simulink model "acf_force_control_simple"  (R2026b)
settings: Solver=ode4  StopTime=4  FixedStep=1.0000000000000001e-05
InitFcn:
  | acf_select_actuator(bdroot);
model workspace (MAT data in the model file):
  acfControlVersion = 'inertial-delivery-v8'
  acfImplementation = 'simple'
  acfLayoutVersion = 1
  p.actuator.kind = 'voice_coil'
  p.sim.step = 1e-05
  p.sim.stopTime = 4
  p.sim.evaluateFrom = 0
  p.force.reference = 50
  p.force.tolerance = 0.5
  p.force.sampleTime = 0.0001
  p.force.antiWindupRate = 30
  p.force.derivativeFilter = 0.001
  p.force.feedforwardEnabled = 1
  p.mechanics.mA = 0.4
  p.mechanics.mB = 0.6
  p.mechanics.mS = 2
  p.mechanics.k1 = 19746
  p.mechanics.k2 = 19746
  p.mechanics.c1 = 60
  p.mechanics.c2 = 0
  p.mechanics.gravity = 9.81
  p.mechanics.angle = 1.57079632679
  p.mechanics.travelMin = 0
  p.mechanics.travelMax = 0.025
  p.mechanics.midTravel = 0.0125
  p.mechanics.lowerRigid = 0
  p.mechanics.upperRigid = 1
  p.mechanics.externalLowerSpringPair = 1
  p.mechanics.externalUpperSpringPair = 0
  p.robot.initialExcessForce = 10
  p.robot.sampleTime = 0.01
  p.robot.delay = 0.08
  p.robot.recenterGain = 0.8
  p.robot.deadband = 0.0005
  p.robot.responseTime = 0.06
  p.robot.maxSpeed = 0.02
  p.robot.maxAcceleration = 0.5
  p.robot.nominalVelocity = 0.005
  p.robot.errorRiseTime = 0.2
  p.robot.errorForce = 20
  p.robot.forceGate.enabled = 1
  p.robot.forceGate.errorBand_N = 0.2
  p.robot.forceGate.maxRate_N_s = 2
  p.robot.forceGate.dwellTime = 0.1
  p.robot.forceGate.filterTime = 0.1
  p.robot.forceGate.maxDelayGainProduct = 0.25
  p.robot.forceGate.variation.enabled = 1
  p.robot.forceGate.variation.meanTime = 0.1
  p.robot.forceGate.variation.varianceTime = 0.02
  p.robot.forceGate.variation.rmsLimit_N = 0.08
  p.robot.initialPositionOffset_m = 0
  p.sensor.sampleTime = 1e-05
  p.sensor.filterTime = 0.0001
  p.sensor.delay = 2e-05
  p.sensor.bias = 0
  p.sensor.noiseRms = 0.02
  p.sensor.seed = 7
  p.sensor.strokeNoiseRms = 1e-06
  p.sensor.strokeDelay = 2e-05
  p.sensor.distalMass_kg = 2
  p.sensor.distalMass_model_kg = 2
  p.sensor.strokeBias = 0
  p.sensor.positionTarget = 'tool_relative_A'
  p.sensor.positionModel = 1
  p.sensor.distalMassCalibrationScale = 1
  p.sensor.lateralDelayOffsetSamples = 0
  p.sensor.strokeDelayOffset_s = 0
  p.surface.kind = 'sharp_bump'
  p.surface.startTime = 2
  p.surface.height = 0.001
  p.surface.width = 0.01
  p.surface.scanSpeed = 0.1
  p.surface.repeatPeriod = 1.2
  p.screw.lead = 0.01
  p.screw.rotorInertia = 1.58e-06
  p.screw.torqueConstant = 0.0234
  p.screw.backEmfConstant = 0.0234
  p.screw.resistance = 2.32
  p.screw.inductance = 0.000238
  p.screw.peakCurrent = 5
  p.screw.voltage = 24
  p.screw.currentResponse = 0.0001
  p.screw.coulombTorque = 0.001
  p.screw.viscousTorque = 1e-06
  p.screw.frictionSpeed = 1
  p.screw.speedBandwidth = 1000
  p.screw.speedDamping = 0.9
  p.screw.speedAntiWindup = 1000
  p.screw.maxLinearSpeedRequest = 0.1
  p.screw.forceKp = 0.0005
  p.screw.forceKi = 0.005
  p.screw.forceKd = 0
  p.screw.motorReference = 'maxon RE25 302005 (NRND): winding reference only'
  p.screw.motorRotorInertia_kg_m2 = 1.08e-06
  p.screw.screwCouplerInertia_kg_m2 = 5e-07
  p.screw.motorMass_kg = 0.13
  p.screw.continuousCurrent_A = 1.16
  p.screw.continuousTorque_Nm = 0.0263
  p.screw.sizingEfficiency = 0.9
  p.screw.currentDerivativeFilter = 0.0003
  p.screw.currentNotch.enabled = 0
  p.screw.currentNotch.frequency_Hz = 20.2167690051
  p.screw.currentNotch.zeroDamping = 0.01
  p.screw.currentNotch.poleDamping = 0.3
  p.screw.feedbackFilter.kind = 'common'
  p.screw.feedbackFilter.zeroDamping = 0.01
  p.screw.feedbackFilter.poleDamping = 0.3
  p.screw.accelerationPrediction_s = 0
  p.screw.accelerationDerivativeFilter_s = 0.0003
  p.screw.accelerationFeedforwardFilter_s = 0
  p.screw.controlStrategy = 'current'
  p.screw.velocityFeedforwardScale = 0
  p.screw.currentForceKp = 0.408089597672
  p.screw.currentForceKi = 27.2059731781
  p.screw.currentForceKd = 0
  p.coil.forceConstant = 20
  p.coil.resistance = 4
  p.coil.inductance = 0.003
  p.coil.peakCurrent = 3.5
  p.coil.voltage = 24
  p.coil.currentResponse = 0.0001
  p.coil.coulombForce = 0.2
  p.coil.viscousFriction = 2
  p.coil.frictionSpeed = 0.0002
  p.coil.strategy = 'pi'
  p.ideal.positionGain = 100
  p.ideal.velocityTime = 0.005
  p.ideal.maxSpeed = 0.1
  p.ideal.maxAcceleration = 20
  p.ideal.maxAxialForce = Inf
  p.ideal.forceKp = 7.49999999996e-05
  p.ideal.forceKi = 0.0179999999999
  p.ideal.forceKd = 0
  p.d.M = 1
  p.d.alpha = 0.4
  p.d.beta = 0.6
  p.d.mu = 0.24
  p.d.g = 6.00689254982e-16
  p.d.keq = 19746
  p.d.ell = 0.00159154943092
  p.d.q10 = 50
  p.d.q20 = 50
  p.d.holdForce = 50
  p.d.r0 = -0.000506431682366
  p.d.u0 = -0.000506431682366
  p.d.z0 = -0.000202572672946
  p.d.forceTicks = 10
  p.d.sensorTicks = 1
  p.d.robotTicks = 1000
  p.d.sensorDelaySamples = 2
  p.d.robotDelaySamples = 800
  p.d.strokeDelaySamples = 2
  p.d.duration = 0.1
  p.d.screwHoldCurrent = 3.40074664726
  p.d.coilHoldCurrent = 2.5
  p.d.speedKp = 0
  p.d.speedKi = 0
  p.d.forceKp = 0.3
  p.d.forceKi = 20
  p.d.forceFeedforward = 2.5
  p.d.commandMax = 3.5
  p.d.commandMin = -3.5
  p.d.recenterGain = 0.735294117647
  p.d.positionMeasurementBias = -0.0130064316824
  p.d.positionMeasurementInitial = 0.0130064316824
  p.d.forceKd = 0
  p.d.derivativeFilter = 0.001
  p.d.toolMotionObserver.A = [0.950360913569  0.0001; -6.16009725429  1]
  p.d.toolMotionObserver.B = [0.0496390864311  5e-09  -5e-09; 6.16009725429  0.0001  -0.0001]
  p.d.toolMotionObserver.C = [0.950976923294  0; -6.16009725429  1]
  p.d.toolMotionObserver.D = [0.0490230767057  0  0; 6.16009725429  0  0]
  p.d.currentNotch.numerator = [1 0 0]
  p.d.currentNotch.denominator = [1 0 0]
  p.d.currentNotch.initialStates = [2.5; 2.5]
  p.d.feedbackFilter.numerator = [0.0674552738891 0.134910547778 0.0674552738891]
  p.d.feedbackFilter.denominator = [1 -1.14298050254 0.412801598096]
  p.d.feedbackFilter.initialStates = [0; 0]
  p.d.variationGate.meanNumerator = [0.000999500166625 0]
  p.d.variationGate.meanDenominator = [1 -0.999000499833]
  p.d.variationGate.varianceNumerator = [0.00498752080732 0]
  p.d.variationGate.varianceDenominator = [1 -0.995012479193]
  p.d.variationGate.dwellSamples = 1001
  p.d.accelerationPrediction.derivativeNumerator = [2834.68689426 -2834.68689426]
  p.d.accelerationPrediction.derivativeDenominator = [1 -0.716531310574]
  p.d.dragRatio.memoryWeight = 0.980198673307
  p.d.dragRatio.inputWeight = 0.0198013266932
  p.d.positionSampleTime = 1e-05
  p.d.acquisition.numerator = [0.00377324111801 0.00754648223602 0.00377324111801 0]
  p.d.acquisition.denominator = [1 -2.37115334916 1.90670140373 -0.520455090097]
  p.d.acquisition.steadyStatePerUnitInput = [66.2560361718; 66.2560361718; 66.2560361718]
  p.d.acquisition.impulseEnergy = 0.0635425312352
  p.d.acquisition.noiseInputScale = 3.96705064105
  p.d.acquisition.rawSampleTime_s = 1e-05
  p.d.acquisition.nominalLowFrequencyDelay_s = 8.89214154824e-05
  p.d.acquisition.responses.force.numerator = [0.00377324111801 0.00754648223602 0.00377324111801 0]
  p.d.acquisition.responses.force.denominator = [1 -2.37115334916 1.90670140373 -0.520455090097]
  p.d.acquisition.responses.force.steadyStatePerUnitInput = [66.2560361718; 66.2560361718; 66.2560361718]
  p.d.acquisition.responses.force.cutoff_Hz = 5100
  p.d.acquisition.responses.force.emaTime_s = 5e-05
  p.d.acquisition.responses.lateral.numerator = [0.00377324111801 0.00754648223602 0.00377324111801 0]
  p.d.acquisition.responses.lateral.denominator = [1 -2.37115334916 1.90670140373 -0.520455090097]
  p.d.acquisition.responses.lateral.steadyStatePerUnitInput = [66.2560361718; 66.2560361718; 66.2560361718]
  p.d.acquisition.responses.lateral.cutoff_Hz = 5100
  p.d.acquisition.responses.lateral.emaTime_s = 5e-05
  p.d.acquisition.responses.acceleration.numerator = [0.00377324111801 0.00754648223602 0.00377324111801 0]
  p.d.acquisition.responses.acceleration.denominator = [1 -2.37115334916 1.90670140373 -0.520455090097]
  p.d.acquisition.responses.acceleration.steadyStatePerUnitInput = [66.2560361718; 66.2560361718; 66.2560361718]
  p.d.acquisition.responses.acceleration.cutoff_Hz = 5100
  p.d.acquisition.responses.acceleration.emaTime_s = 5e-05
  p.d.acquisition.responses.position.numerator = [0.00377324111801 0.00754648223602 0.00377324111801 0]
  p.d.acquisition.responses.position.denominator = [1 -2.37115334916 1.90670140373 -0.520455090097]
  p.d.acquisition.responses.position.steadyStatePerUnitInput = [66.2560361718; 66.2560361718; 66.2560361718]
  p.d.acquisition.responses.position.cutoff_Hz = 5100
  p.d.acquisition.responses.position.emaTime_s = 5e-05
  p.d.acquisition.responses.frame.numerator = [0.00377324111801 0.00754648223602 0.00377324111801 0]
  p.d.acquisition.responses.frame.denominator = [1 -2.37115334916 1.90670140373 -0.520455090097]
  p.d.acquisition.responses.frame.steadyStatePerUnitInput = [66.2560361718; 66.2560361718; 66.2560361718]
  p.d.acquisition.responses.frame.cutoff_Hz = 5100
  p.d.acquisition.responses.frame.emaTime_s = 5e-05
  p.d.acquisition.noiseReferenceImpulseEnergy = 0.0635425312352
  p.d.acquisition.frameDelaySamples = 2
  p.d.acquisition.accelerationNoiseInputScale = 3.96705064105
  p.d.acquisition.positionNoiseInputScale = 3.96705064105
  p.d.actualRobotTransportSampleTime_s = 0.0001
  p.d.preparedScanSpeed_m_s = 0.1
  p.d.preparedSensorDelay_s = 2e-05
  p.d.identifiedHolderMass_kg = 0.6
  p.d.identifiedMovingMass_kg = 2.6
  p.d.coilForceConstant_model_N_A = 20
  p.d.screwTorqueConstant_model_Nm_A = 0.0234
  p.d.coilHoldingCurrentCommand_A = 2.5
  p.d.screwHoldingCurrentCommand_A = 3.40074664726
  p.d.screwMovingMass = 0.6
  p.d.screwAccelerationPrediction.derivativeNumerator = [2834.68689426 -2834.68689426]
  p.d.screwAccelerationPrediction.derivativeDenominator = [1 -0.716531310574]
  p.d.screwAccelerationFeedforwardFilter.numerator = [1 0]
  p.d.screwAccelerationFeedforwardFilter.denominator = [1 0]
  p.d.screwCurrentNotch.numerator = [1 0 0]
  p.d.screwCurrentNotch.denominator = [1 0 0]
  p.d.screwCurrentNotch.initialStates = [3.40074664726; 3.40074664726]
  p.d.screwFeedbackFilter.numerator = [0.0674552738891 0.134910547778 0.0674552738891]
  p.d.screwFeedbackFilter.denominator = [1 -1.14298050254 0.412801598096]
  p.d.screwFeedbackFilter.initialStates = [0; 0]
  p.d.screwLowerLoadInverse.enabled = 1
  p.d.screwLowerLoadInverse.scale = 1
  p.d.screwLowerLoadInverse.cutoff_Hz = 1500
  p.d.screwLowerLoadInverse.filterDamping = 0.707106781187
  p.d.screwLowerLoadInverse.identifiedStiffness_N_m = 19746
  p.d.screwLowerLoadInverse.identifiedDamping_Ns_m = 60
  p.d.screwLowerLoadInverse.identifiedMassB_kg = 1.22375899815
  p.d.screwLowerLoadInverse.numerator = [3.57861341628 -3.57861341628 -3.57861341628 3.57861341628]
  p.d.screwLowerLoadInverse.denominator = [1 -1.71541194562 0.995792771996 -0.263401371553]
  p.d.screwLowerLoadInverse.identifiedForceConstant_N_A = 14.7026536188
  p.d.screwLowerLoadInverse.stiffnessCalibrationScale = 1
  p.d.screwLowerLoadInverse.dampingCalibrationScale = 1
  p.d.screwLowerLoadInverse.dampingCalibrationOffset_Ns_m = 0
  p.robotPrediction.enabled = 1
  p.robotPrediction.delay = 0.08
  p.robotPrediction.responseTime = 0.06
  p.robotPrediction.maxSpeed = 0.02
  p.robotPrediction.maxAcceleration = 0.5
  p.robotPrediction.boundedNominalPath = 1
  p.robotPrediction.delaySamples = 8
  p.robotPrediction.surfaceJerkEnabled = 0
  p.robotPrediction.surfaceSnapPower = 1000000
  p.robotPrediction.surfaceJerkDecayTime = Inf
  p.robotPrediction.surfaceJerkFeedforwardGain = 0
  p.contact.mu = 0.3
  p.contact.lateralNoiseRms_N = 0.02
  p.contact.lateralBias_N = 0
  p.contact.slopeFilterTime_s = 0
  p.contact.normalIntegralScale = 1
  p.contact.geometryFeedforwardScale = 1
  p.contact.lateralPredictionTime_s = 0
  p.contact.lateralDerivativeFilterTime_s = 0.0003
  p.contact.commandedScanSpeed_m_s = 0.1
  p.contact.lateralDelaySamples = 2
  p.contact.geometryMode = 'measured_drag_ratio'
  p.contact.dragRatioFilter_s = 0.005
  p.contact.dragRatioMinForce_N = 1
  p.contact.commandedScanSpeedScale = 1
  p.accel.enabled = 1
  p.accel.filterTime = 0.0001
  p.accel.delay = 2e-05
  p.accel.noiseRms = 0.014
  p.accel.bias = 0
  p.accel.scaleError = 0
  p.accel.range_g = 50
  p.accel.quantum = 0.00468
  p.accel.delaySamples = 2
  p.accel.nominalNoiseRms = 0.014
  p.accel.delayOffset_s = 0
  p.inertial.forceKp = 0.3
  p.inertial.forceKi = 20
  p.inertial.forceKd = 0
  p.inertial.derivativeFilter = 0.001
  p.inertial.positionBandwidth_Hz = 40
  p.inertial.accelerationFeedforwardScale = 1
  p.inertial.guideFrictionFeedforwardScale = 1
  p.inertial.guideVelocityPrediction_s = 0.0004
  p.inertial.currentNotch.enabled = 0
  p.inertial.currentNotch.frequency_Hz = 1643.74518416
  p.inertial.currentNotch.zeroDamping = 0.001
  p.inertial.currentNotch.poleDamping = 1
  p.inertial.feedbackFilter.enabled = 1
  p.inertial.feedbackFilter.cutoff_Hz = 1000
  p.inertial.feedbackFilter.damping = 0.707106781187
  p.inertial.accelerationPrediction_s = 0
  p.inertial.accelerationDerivativeFilter_s = 0.0003
  p.inertial.lowerLoadInverse.enabled = 1
  p.inertial.lowerLoadInverse.scale = 1
  p.inertial.lowerLoadInverse.cutoff_Hz = 1500
  p.inertial.lowerLoadInverse.filterDamping = 0.707106781187
  p.inertial.lowerLoadInverse.identifiedStiffness_N_m = 19746
  p.inertial.lowerLoadInverse.identifiedDamping_Ns_m = 60
  p.inertial.lowerLoadInverse.identifiedMassB_kg = 0.6
  p.inertial.lowerLoadInverse.numerator = [1.28984008064 -1.28984008064 -1.28984008064 1.28984008064]
  p.inertial.lowerLoadInverse.denominator = [1 -1.71541194562 0.995792771996 -0.263401371553]
  p.inertial.lowerLoadInverse.identifiedForceConstant_N_A = 20
  p.inertial.lowerLoadInverse.stiffnessCalibrationScale = 1
  p.inertial.lowerLoadInverse.dampingCalibrationScale = 1
  p.inertial.lowerLoadInverse.dampingCalibrationOffset_Ns_m = 0
  p.inertial.holderMassCalibrationScale = 1
  p.inertial.forceConstantCalibrationScale = 1
  p.sensorDesign.accelerometer = 'Two orthogonal ADXL1002 analog axes'
  p.sensorDesign.noiseDensity_ug_sqrtHz = 25
  p.sensorDesign.assumedENBW_Hz = 3177.12656176
  p.sensorDesign.derivedRMS_m_s2 = 0.0138190421649
  p.sensorDesign.modeledRMS_m_s2 = 0.014
  p.sensorDesign.nominalModeledRMS_m_s2 = 0.014
  p.sensorDesign.ADCbits = 18
  p.sensorDesign.ADCvoltageRange_V = [0 5]
  p.sensorDesign.sensitivity_V_g = 0.04
  p.sensorDesign.derivedQuantum_m_s2 = 0.00467617511749
  p.sensorDesign.modeledQuantum_m_s2 = 0.00468
  p.sensorDesign.modeledRange_g = 50
  p.sensorDesign.rawSampleTime_s = 1e-05
  p.sensorDesign.antiAliasCutoff_Hz = 5100
  p.sensorDesign.antiAliasDamping = 0.707106781187
  p.sensorDesign.conditioningEMA_s = 5e-05
  p.sensorDesign.responseGroupDelay_s = 8.89214154824e-05
  p.sensorDesign.commonAcquisitionDelay_s = 2e-05
  p.sensorDesign.identifiedMotionFrameDelay_s = 2e-05
  p.sensorDesign.forceConditioning = 'Designed common two-pole AA and fresh EMA; actual and identified response/phase are explicit.'
  p.sensorDesign.interpretation = 'Engineered and identified acquisition target, not a guaranteed manufacturer transfer. Noise is conditioned RMS before conservative post-response ADC quantization.'
  p.springs.lower.part = 'Approximate guided spring target; confirm working envelope'
  p.springs.lower.rate_N_m = 9873
  p.springs.lower.freeLength_m = 0.02
  p.springs.lower.freeLengthTolerance_m = 0.00049
  p.springs.lower.minWorkingLength_m = 0.01055
  p.springs.lower.maxCyclicStroke_m = 0.00318
  p.springs.lower.forceEnvelope_N = 68.543
  p.springs.upper.part = 'Approximate guided spring target; confirm working envelope'
  p.springs.upper.rate_N_m = 9873
  p.springs.upper.freeLength_m = 0.02
  p.springs.upper.freeLengthTolerance_m = 0.00049
  p.springs.upper.minWorkingLength_m = 0.01055
  p.springs.upper.maxCyclicStroke_m = 0.00318
  p.springs.upper.forceEnvelope_N = 68.543
  p.springs.commonPreload_N = 33.6
  p.springs.maxCombinedLength_m = 0.1
  p.springs.workingClearance_m = 0.0005
  p.springs.unseatingClearance_m = 0.00025
  p.springs.sensingCell.stiffness_N_m = 64000000
  p.springs.sensingCell.separateNativeState = 0
  p.springs.sensingCell.masslessSeriesApproximation = 1
  p.springs.sensingCell.structuralDampingQualified = 0
  p.springs.sensingCell.loadPath = 'B -> opposed guided spring pair parallel with damper -> joining frame -> multi-axis B-S load cell -> S'
  p.springs.sensingCell.loadCellBypass = 0
  p.springs.sensingCell.prototypeMountModeQualificationRequired = 1
  p.acquisition.enabled = 1
  p.acquisition.rawSampleTime_s = 1e-05
  p.acquisition.antiAliasCutoff_Hz = 5100
  p.acquisition.antiAliasDamping = 0.707106781187
  p.acquisition.emaTime_s = 5e-05
  p.acquisition.pipelineDelay_s = 2e-05
  p.acquisition.forceDelayOffset_s = 0
  p.acquisition.lateralDelayOffset_s = 0
  p.acquisition.accelerationDelayOffset_s = 0
  p.acquisition.positionDelayOffset_s = 0
  p.acquisition.requireFastVariationGate = 1
  p.acquisition.identifiedAntiAliasCutoff_Hz = 5100
  p.acquisition.identifiedEmaTime_s = 5e-05
  p.acquisition.identifiedPipelineDelay_s = 2e-05
  p.acquisition.forceAntiAliasScale = 1
  p.acquisition.lateralAntiAliasScale = 1
  p.acquisition.accelerationAntiAliasScale = 1
  p.acquisition.positionAntiAliasScale = 1
  p.acquisition.motionFrameDelayOffset_s = 0
  pCompliant.actuator.kind = 'voice_coil'
  pCompliant.sim.step = 1e-05
  pCompliant.sim.stopTime = 4
  pCompliant.sim.evaluateFrom = 0
  pCompliant.force.reference = 50
  pCompliant.force.tolerance = 0.5
  pCompliant.force.sampleTime = 0.0001
  pCompliant.force.antiWindupRate = 30
  pCompliant.force.derivativeFilter = 0.001
  pCompliant.force.feedforwardEnabled = 1
  pCompliant.mechanics.mA = 0.4
  pCompliant.mechanics.mB = 0.6
  pCompliant.mechanics.mS = 1.4
  pCompliant.mechanics.k1 = 19746
  pCompliant.mechanics.k2 = 19746
  pCompliant.mechanics.c1 = 30
  pCompliant.mechanics.c2 = 5
  pCompliant.mechanics.gravity = 9.81
  pCompliant.mechanics.angle = 0
  pCompliant.mechanics.travelMin = 0
  pCompliant.mechanics.travelMax = 0.025
  pCompliant.mechanics.midTravel = 0.0125
  pCompliant.mechanics.lowerRigid = 0
  pCompliant.mechanics.upperRigid = 0
  pCompliant.mechanics.externalLowerSpringPair = 1
  pCompliant.mechanics.externalUpperSpringPair = 1
  pCompliant.robot.initialExcessForce = 10
  pCompliant.robot.sampleTime = 0.01
  pCompliant.robot.delay = 0.08
  pCompliant.robot.recenterGain = 0.8
  pCompliant.robot.deadband = 0.0005
  pCompliant.robot.responseTime = 0.06
  pCompliant.robot.maxSpeed = 0.02
  pCompliant.robot.maxAcceleration = 0.5
  pCompliant.robot.nominalVelocity = 0.005
  pCompliant.robot.errorRiseTime = 0.2
  pCompliant.robot.errorForce = 20
  pCompliant.robot.forceGate.enabled = 1
  pCompliant.robot.forceGate.errorBand_N = 0.2
  pCompliant.robot.forceGate.maxRate_N_s = 2
  pCompliant.robot.forceGate.dwellTime = 0.1
  pCompliant.robot.forceGate.filterTime = 0.1
  pCompliant.robot.forceGate.maxDelayGainProduct = 0.25
  pCompliant.robot.forceGate.variation.enabled = 1
  pCompliant.robot.forceGate.variation.meanTime = 0.1
  pCompliant.robot.forceGate.variation.varianceTime = 0.02
  pCompliant.robot.forceGate.variation.rmsLimit_N = 0.08
  pCompliant.robot.initialPositionOffset_m = 0
  pCompliant.sensor.sampleTime = 1e-05
  pCompliant.sensor.filterTime = 0.0001
  pCompliant.sensor.delay = 2e-05
  pCompliant.sensor.bias = 0
  pCompliant.sensor.noiseRms = 0.02
  pCompliant.sensor.seed = 7
  pCompliant.sensor.strokeNoiseRms = 1e-06
  pCompliant.sensor.strokeDelay = 2e-05
  pCompliant.sensor.distalMass_kg = 1.4
  pCompliant.sensor.distalMass_model_kg = 1.4
  pCompliant.sensor.strokeBias = 0
  pCompliant.sensor.positionTarget = 'tool_relative_A'
  pCompliant.sensor.positionModel = 1
  pCompliant.sensor.distalMassCalibrationScale = 1
  pCompliant.sensor.lateralDelayOffsetSamples = 0
  pCompliant.sensor.strokeDelayOffset_s = 0
  pCompliant.surface.kind = 'sharp_bump'
  pCompliant.surface.startTime = 2
  pCompliant.surface.height = 0.001
  pCompliant.surface.width = 0.01
  pCompliant.surface.scanSpeed = 0.1
  pCompliant.surface.repeatPeriod = 1.2
  pCompliant.screw.lead = 0.01
  pCompliant.screw.rotorInertia = 1.58e-06
  pCompliant.screw.torqueConstant = 0.0234
  pCompliant.screw.backEmfConstant = 0.0234
  pCompliant.screw.resistance = 2.32
  pCompliant.screw.inductance = 0.000238
  pCompliant.screw.peakCurrent = 5
  pCompliant.screw.voltage = 24
  pCompliant.screw.currentResponse = 0.0001
  pCompliant.screw.coulombTorque = 0.001
  pCompliant.screw.viscousTorque = 1e-06
  pCompliant.screw.frictionSpeed = 1
  pCompliant.screw.speedBandwidth = 1000
  pCompliant.screw.speedDamping = 0.9
  pCompliant.screw.speedAntiWindup = 1000
  pCompliant.screw.maxLinearSpeedRequest = 0.1
  pCompliant.screw.forceKp = 0.0005
  pCompliant.screw.forceKi = 0.005
  pCompliant.screw.forceKd = 0
  pCompliant.screw.motorReference = 'maxon RE25 302005 (NRND): winding reference only'
  pCompliant.screw.motorRotorInertia_kg_m2 = 1.08e-06
  pCompliant.screw.screwCouplerInertia_kg_m2 = 5e-07
  pCompliant.screw.motorMass_kg = 0.13
  pCompliant.screw.continuousCurrent_A = 1.16
  pCompliant.screw.continuousTorque_Nm = 0.0263
  pCompliant.screw.sizingEfficiency = 0.9
  pCompliant.screw.currentDerivativeFilter = 0.0003
  pCompliant.screw.currentNotch.enabled = 0
  pCompliant.screw.currentNotch.frequency_Hz = 20.2167690051
  pCompliant.screw.currentNotch.zeroDamping = 0.01
  pCompliant.screw.currentNotch.poleDamping = 0.3
  pCompliant.screw.feedbackFilter.kind = 'common'
  pCompliant.screw.feedbackFilter.zeroDamping = 0.01
  pCompliant.screw.feedbackFilter.poleDamping = 0.3
  pCompliant.screw.accelerationPrediction_s = 0
  pCompliant.screw.accelerationDerivativeFilter_s = 0.0003
  pCompliant.screw.accelerationFeedforwardFilter_s = 0
  pCompliant.screw.controlStrategy = 'current'
  pCompliant.screw.velocityFeedforwardScale = 0
  pCompliant.screw.currentForceKp = 0.408089597672
  pCompliant.screw.currentForceKi = 27.2059731781
  pCompliant.screw.currentForceKd = 0
  pCompliant.coil.forceConstant = 20
  pCompliant.coil.resistance = 4
  pCompliant.coil.inductance = 0.003
  pCompliant.coil.peakCurrent = 3.5
  pCompliant.coil.voltage = 24
  pCompliant.coil.currentResponse = 0.0001
  pCompliant.coil.coulombForce = 0.2
  pCompliant.coil.viscousFriction = 2
  pCompliant.coil.frictionSpeed = 0.0002
  pCompliant.coil.strategy = 'pi'
  pCompliant.ideal.positionGain = 100
  pCompliant.ideal.velocityTime = 0.005
  pCompliant.ideal.maxSpeed = 0.1
  pCompliant.ideal.maxAcceleration = 20
  pCompliant.ideal.maxAxialForce = Inf
  pCompliant.ideal.forceKp = 7.49999999996e-05
  pCompliant.ideal.forceKi = 0.0179999999999
  pCompliant.ideal.forceKd = 0
  pCompliant.d.M = 1
  pCompliant.d.alpha = 0.4
  pCompliant.d.beta = 0.6
  pCompliant.d.mu = 0.24
  pCompliant.d.g = 9.81
  pCompliant.d.keq = 9873
  pCompliant.d.ell = 0.00159154943092
  pCompliant.d.q10 = 36.266
  pCompliant.d.q20 = 26.456
  pCompliant.d.holdForce = 30.38
  pCompliant.d.r0 = -0.00101286336473
  pCompliant.d.u0 = -0.00101286336473
  pCompliant.d.z0 = -0.000405145345893
  pCompliant.d.forceTicks = 10
  pCompliant.d.sensorTicks = 1
  pCompliant.d.robotTicks = 1000
  pCompliant.d.sensorDelaySamples = 2
  pCompliant.d.robotDelaySamples = 800
  pCompliant.d.strokeDelaySamples = 2
  pCompliant.d.duration = 0.1
  pCompliant.d.screwHoldCurrent = 2.06629366288
  pCompliant.d.coilHoldCurrent = 1.519
  pCompliant.d.speedKp = 0
  pCompliant.d.speedKi = 0
  pCompliant.d.forceKp = 0.3
  pCompliant.d.forceKi = 20
  pCompliant.d.forceFeedforward = 1.519
  pCompliant.d.commandMax = 3.5
  pCompliant.d.commandMin = -3.5
  pCompliant.d.recenterGain = 0.735294117647
  pCompliant.d.positionMeasurementBias = -0.0135128633647
  pCompliant.d.positionMeasurementInitial = 0.0135128633647
  pCompliant.d.forceKd = 0
  pCompliant.d.derivativeFilter = 0.001
  pCompliant.d.positionSampleTime = 1e-05
  pCompliant.d.actualRobotTransportSampleTime_s = 0.0001
  pCompliant.d.preparedScanSpeed_m_s = 0.1
  pCompliant.d.preparedSensorDelay_s = 2e-05
  pCompliant.d.identifiedHolderMass_kg = 0.6
  pCompliant.d.identifiedMovingMass_kg = 2
  pCompliant.d.coilForceConstant_model_N_A = 20
  pCompliant.d.screwTorqueConstant_model_Nm_A = 0.0234
  pCompliant.d.coilHoldingCurrentCommand_A = 1.519
  pCompliant.d.screwHoldingCurrentCommand_A = 2.06629366288
  pCompliant.d.screwMovingMass = 0.24
  pCompliant.d.screwAccelerationPrediction.derivativeNumerator = [2834.68689426 -2834.68689426]
  pCompliant.d.screwAccelerationPrediction.derivativeDenominator = [1 -0.716531310574]
  pCompliant.d.screwAccelerationFeedforwardFilter.numerator = [1 0]
  pCompliant.d.screwAccelerationFeedforwardFilter.denominator = [1 0]
  pCompliant.d.screwCurrentNotch.numerator = [1 0 0]
  pCompliant.d.screwCurrentNotch.denominator = [1 0 0]
  pCompliant.d.screwCurrentNotch.initialStates = [2.06629366288; 2.06629366288]
  pCompliant.d.screwFeedbackFilter.numerator = [0.0674552738891 0.134910547778 0.0674552738891]
  pCompliant.d.screwFeedbackFilter.denominator = [1 -1.14298050254 0.412801598096]
  pCompliant.d.screwFeedbackFilter.initialStates = [0; 0]
  pCompliant.d.screwLowerLoadInverse.enabled = 1
  pCompliant.d.screwLowerLoadInverse.scale = 1
  pCompliant.d.screwLowerLoadInverse.cutoff_Hz = 1500
  pCompliant.d.screwLowerLoadInverse.filterDamping = 0.707106781187
  pCompliant.d.screwLowerLoadInverse.identifiedStiffness_N_m = 19746
  pCompliant.d.screwLowerLoadInverse.identifiedDamping_Ns_m = 30
  pCompliant.d.screwLowerLoadInverse.identifiedMassB_kg = 1.22375899815
  pCompliant.d.screwLowerLoadInverse.numerator = [7.04320705588 -7.04320705588 -7.04320705588 7.04320705588]
  pCompliant.d.screwLowerLoadInverse.denominator = [1 -1.68406629824 0.972352836098 -0.254868618096]
  pCompliant.d.screwLowerLoadInverse.identifiedForceConstant_N_A = 14.7026536188
  pCompliant.d.screwLowerLoadInverse.stiffnessCalibrationScale = 1
  pCompliant.d.screwLowerLoadInverse.dampingCalibrationScale = 1
  pCompliant.d.screwLowerLoadInverse.dampingCalibrationOffset_Ns_m = 0
  pCompliant.d.currentNotch.numerator = [1 0 0]
  pCompliant.d.currentNotch.denominator = [1 0 0]
  pCompliant.d.currentNotch.initialStates = [1.519; 1.519]
  pCompliant.d.feedbackFilter.numerator = [0.0674552738891 0.134910547778 0.0674552738891]
  pCompliant.d.feedbackFilter.denominator = [1 -1.14298050254 0.412801598096]
  pCompliant.d.feedbackFilter.initialStates = [0; 0]
  pCompliant.d.variationGate.meanNumerator = [0.000999500166625 0]
  pCompliant.d.variationGate.meanDenominator = [1 -0.999000499833]
  pCompliant.d.variationGate.varianceNumerator = [0.00498752080732 0]
  pCompliant.d.variationGate.varianceDenominator = [1 -0.995012479193]
  pCompliant.d.variationGate.dwellSamples = 1001
  pCompliant.d.accelerationPrediction.derivativeNumerator = [2834.68689426 -2834.68689426]
  pCompliant.d.accelerationPrediction.derivativeDenominator = [1 -0.716531310574]
  pCompliant.d.dragRatio.memoryWeight = 0.980198673307
  pCompliant.d.dragRatio.inputWeight = 0.0198013266932
  pCompliant.d.toolMotionObserver.A = [0.950360913569  0.0001; -6.16009725429  1]
  pCompliant.d.toolMotionObserver.B = [0.0496390864311  5e-09  -5e-09; 6.16009725429  0.0001  -0.0001]
  pCompliant.d.toolMotionObserver.C = [0.950976923294  0; -6.16009725429  1]
  pCompliant.d.toolMotionObserver.D = [0.0490230767057  0  0; 6.16009725429  0  0]
  pCompliant.d.acquisition.numerator = [0.00377324111801 0.00754648223602 0.00377324111801 0]
  pCompliant.d.acquisition.denominator = [1 -2.37115334916 1.90670140373 -0.520455090097]
  pCompliant.d.acquisition.steadyStatePerUnitInput = [66.2560361718; 66.2560361718; 66.2560361718]
  pCompliant.d.acquisition.impulseEnergy = 0.0635425312352
  pCompliant.d.acquisition.noiseInputScale = 3.96705064105
  pCompliant.d.acquisition.rawSampleTime_s = 1e-05
  pCompliant.d.acquisition.nominalLowFrequencyDelay_s = 8.89214154824e-05
  pCompliant.d.acquisition.responses.force.numerator = [0.00377324111801 0.00754648223602 0.00377324111801 0]
  pCompliant.d.acquisition.responses.force.denominator = [1 -2.37115334916 1.90670140373 -0.520455090097]
  pCompliant.d.acquisition.responses.force.steadyStatePerUnitInput = [66.2560361718; 66.2560361718; 66.2560361718]
  pCompliant.d.acquisition.responses.force.cutoff_Hz = 5100
  pCompliant.d.acquisition.responses.force.emaTime_s = 5e-05
  pCompliant.d.acquisition.responses.lateral.numerator = [0.00377324111801 0.00754648223602 0.00377324111801 0]
  pCompliant.d.acquisition.responses.lateral.denominator = [1 -2.37115334916 1.90670140373 -0.520455090097]
  pCompliant.d.acquisition.responses.lateral.steadyStatePerUnitInput = [66.2560361718; 66.2560361718; 66.2560361718]
  pCompliant.d.acquisition.responses.lateral.cutoff_Hz = 5100
  pCompliant.d.acquisition.responses.lateral.emaTime_s = 5e-05
  pCompliant.d.acquisition.responses.acceleration.numerator = [0.00377324111801 0.00754648223602 0.00377324111801 0]
  pCompliant.d.acquisition.responses.acceleration.denominator = [1 -2.37115334916 1.90670140373 -0.520455090097]
  pCompliant.d.acquisition.responses.acceleration.steadyStatePerUnitInput = [66.2560361718; 66.2560361718; 66.2560361718]
  pCompliant.d.acquisition.responses.acceleration.cutoff_Hz = 5100
  pCompliant.d.acquisition.responses.acceleration.emaTime_s = 5e-05
  pCompliant.d.acquisition.responses.position.numerator = [0.00377324111801 0.00754648223602 0.00377324111801 0]
  pCompliant.d.acquisition.responses.position.denominator = [1 -2.37115334916 1.90670140373 -0.520455090097]
  pCompliant.d.acquisition.responses.position.steadyStatePerUnitInput = [66.2560361718; 66.2560361718; 66.2560361718]
  pCompliant.d.acquisition.responses.position.cutoff_Hz = 5100
  pCompliant.d.acquisition.responses.position.emaTime_s = 5e-05
  pCompliant.d.acquisition.responses.frame.numerator = [0.00377324111801 0.00754648223602 0.00377324111801 0]
  pCompliant.d.acquisition.responses.frame.denominator = [1 -2.37115334916 1.90670140373 -0.520455090097]
  pCompliant.d.acquisition.responses.frame.steadyStatePerUnitInput = [66.2560361718; 66.2560361718; 66.2560361718]
  pCompliant.d.acquisition.responses.frame.cutoff_Hz = 5100
  pCompliant.d.acquisition.responses.frame.emaTime_s = 5e-05
  pCompliant.d.acquisition.noiseReferenceImpulseEnergy = 0.0635425312352
  pCompliant.d.acquisition.frameDelaySamples = 2
  pCompliant.d.acquisition.accelerationNoiseInputScale = 3.96705064105
  pCompliant.d.acquisition.positionNoiseInputScale = 3.96705064105
  pCompliant.springs.maxCombinedLength_m = 0.1
  pCompliant.springs.commonPreload_N = 34
  pCompliant.springs.workingClearance_m = 0.0005
  pCompliant.springs.unseatingClearance_m = 0.00025
  pCompliant.springs.lower.part = 'D-180S'
  pCompliant.springs.lower.rate_N_m = 9873
  pCompliant.springs.lower.freeLength_m = 0.0181
  pCompliant.springs.lower.freeLengthTolerance_m = 0.00049
  pCompliant.springs.lower.minWorkingLength_m = 0.01055
  pCompliant.springs.lower.maxCyclicStroke_m = 0.00318
  pCompliant.springs.lower.forceEnvelope_N = 68.543
  pCompliant.springs.upper.part = 'D-180S'
  pCompliant.springs.upper.rate_N_m = 9873
  pCompliant.springs.upper.freeLength_m = 0.0181
  pCompliant.springs.upper.freeLengthTolerance_m = 0.00049
  pCompliant.springs.upper.minWorkingLength_m = 0.01055
  pCompliant.springs.upper.maxCyclicStroke_m = 0.00318
  pCompliant.springs.upper.forceEnvelope_N = 68.543
  pCompliant.robotPrediction.enabled = 1
  pCompliant.robotPrediction.delay = 0.08
  pCompliant.robotPrediction.responseTime = 0.06
  pCompliant.robotPrediction.maxSpeed = 0.02
  pCompliant.robotPrediction.maxAcceleration = 0.5
  pCompliant.robotPrediction.boundedNominalPath = 1
  pCompliant.robotPrediction.delaySamples = 8
  pCompliant.robotPrediction.surfaceJerkEnabled = 0
  pCompliant.robotPrediction.surfaceSnapPower = 1000000
  pCompliant.robotPrediction.surfaceJerkDecayTime = Inf
  pCompliant.robotPrediction.surfaceJerkFeedforwardGain = 0
  pCompliant.contact.mu = 0.3
  pCompliant.contact.lateralNoiseRms_N = 0.02
  pCompliant.contact.lateralBias_N = 0
  pCompliant.contact.slopeFilterTime_s = 0
  pCompliant.contact.normalIntegralScale = 1
  pCompliant.contact.geometryFeedforwardScale = 1
  pCompliant.contact.lateralPredictionTime_s = 0
  pCompliant.contact.lateralDerivativeFilterTime_s = 0.0003
  pCompliant.contact.commandedScanSpeed_m_s = 0.1
  pCompliant.contact.lateralDelaySamples = 2
  pCompliant.contact.geometryMode = 'measured_drag_ratio'
  pCompliant.contact.dragRatioFilter_s = 0.005
  pCompliant.contact.dragRatioMinForce_N = 1
  pCompliant.contact.commandedScanSpeedScale = 1
  pCompliant.accel.enabled = 1
  pCompliant.accel.filterTime = 0.0001
  pCompliant.accel.delay = 2e-05
  pCompliant.accel.noiseRms = 0.014
  pCompliant.accel.bias = 0
  pCompliant.accel.scaleError = 0
  pCompliant.accel.range_g = 50
  pCompliant.accel.quantum = 0.00468
  pCompliant.accel.delaySamples = 2
  pCompliant.accel.nominalNoiseRms = 0.014
  pCompliant.accel.delayOffset_s = 0
  pCompliant.inertial.forceKp = 0.3
  pCompliant.inertial.forceKi = 20
  pCompliant.inertial.forceKd = 0
  pCompliant.inertial.derivativeFilter = 0.001
  pCompliant.inertial.positionBandwidth_Hz = 40
  pCompliant.inertial.accelerationFeedforwardScale = 1
  pCompliant.inertial.guideFrictionFeedforwardScale = 1
  pCompliant.inertial.guideVelocityPrediction_s = 0.0004
  pCompliant.inertial.currentNotch.enabled = 0
  pCompliant.inertial.currentNotch.frequency_Hz = 1643.74518416
  pCompliant.inertial.currentNotch.zeroDamping = 0.001
  pCompliant.inertial.currentNotch.poleDamping = 1
  pCompliant.inertial.feedbackFilter.enabled = 1
  pCompliant.inertial.feedbackFilter.cutoff_Hz = 1000
  pCompliant.inertial.feedbackFilter.damping = 0.707106781187
  pCompliant.inertial.accelerationPrediction_s = 0
  pCompliant.inertial.accelerationDerivativeFilter_s = 0.0003
  pCompliant.inertial.lowerLoadInverse.enabled = 1
  pCompliant.inertial.lowerLoadInverse.scale = 1
  pCompliant.inertial.lowerLoadInverse.cutoff_Hz = 1500
  pCompliant.inertial.lowerLoadInverse.filterDamping = 0.707106781187
  pCompliant.inertial.lowerLoadInverse.identifiedStiffness_N_m = 19746
  pCompliant.inertial.lowerLoadInverse.identifiedDamping_Ns_m = 30
  pCompliant.inertial.lowerLoadInverse.identifiedMassB_kg = 0.6
  pCompliant.inertial.lowerLoadInverse.numerator = [2.53858399893 -2.53858399893 -2.53858399893 2.53858399893]
  pCompliant.inertial.lowerLoadInverse.denominator = [1 -1.68406629824 0.972352836098 -0.254868618096]
  pCompliant.inertial.lowerLoadInverse.identifiedForceConstant_N_A = 20
  pCompliant.inertial.lowerLoadInverse.stiffnessCalibrationScale = 1
  pCompliant.inertial.lowerLoadInverse.dampingCalibrationScale = 1
  pCompliant.inertial.lowerLoadInverse.dampingCalibrationOffset_Ns_m = 0
  pCompliant.inertial.holderMassCalibrationScale = 1
  pCompliant.inertial.forceConstantCalibrationScale = 1
  pCompliant.acquisition.enabled = 1
  pCompliant.acquisition.rawSampleTime_s = 1e-05
  pCompliant.acquisition.antiAliasCutoff_Hz = 5100
  pCompliant.acquisition.antiAliasDamping = 0.707106781187
  pCompliant.acquisition.emaTime_s = 5e-05
  pCompliant.acquisition.pipelineDelay_s = 2e-05
  pCompliant.acquisition.forceDelayOffset_s = 0
  pCompliant.acquisition.lateralDelayOffset_s = 0
  pCompliant.acquisition.accelerationDelayOffset_s = 0
  pCompliant.acquisition.positionDelayOffset_s = 0
  pCompliant.acquisition.requireFastVariationGate = 1
  pCompliant.acquisition.identifiedAntiAliasCutoff_Hz = 5100
  pCompliant.acquisition.identifiedEmaTime_s = 5e-05
  pCompliant.acquisition.identifiedPipelineDelay_s = 2e-05
  pCompliant.acquisition.forceAntiAliasScale = 1
  pCompliant.acquisition.lateralAntiAliasScale = 1
  pCompliant.acquisition.accelerationAntiAliasScale = 1
  pCompliant.acquisition.positionAntiAliasScale = 1
  pCompliant.acquisition.motionFrameDelayOffset_s = 0
  pCompliant.sensorDesign.accelerometer = 'Two orthogonal ADXL1002 analog axes'
  pCompliant.sensorDesign.noiseDensity_ug_sqrtHz = 25
  pCompliant.sensorDesign.assumedENBW_Hz = 3177.12656176
  pCompliant.sensorDesign.derivedRMS_m_s2 = 0.0138190421649
  pCompliant.sensorDesign.modeledRMS_m_s2 = 0.014
  pCompliant.sensorDesign.nominalModeledRMS_m_s2 = 0.014
  pCompliant.sensorDesign.ADCbits = 18
  pCompliant.sensorDesign.ADCvoltageRange_V = [0 5]
  pCompliant.sensorDesign.sensitivity_V_g = 0.04
  pCompliant.sensorDesign.derivedQuantum_m_s2 = 0.00467617511749
  pCompliant.sensorDesign.modeledQuantum_m_s2 = 0.00468
  pCompliant.sensorDesign.modeledRange_g = 50
  pCompliant.sensorDesign.rawSampleTime_s = 1e-05
  pCompliant.sensorDesign.antiAliasCutoff_Hz = 5100
  pCompliant.sensorDesign.antiAliasDamping = 0.707106781187
  pCompliant.sensorDesign.conditioningEMA_s = 5e-05
  pCompliant.sensorDesign.responseGroupDelay_s = 8.89214154824e-05
  pCompliant.sensorDesign.commonAcquisitionDelay_s = 2e-05
  pCompliant.sensorDesign.identifiedMotionFrameDelay_s = 2e-05
  pCompliant.sensorDesign.forceConditioning = 'Designed common two-pole AA and fresh EMA; actual and identified response/phase are explicit.'
  pCompliant.sensorDesign.interpretation = 'Engineered and identified acquisition target, not a guaranteed manufacturer transfer. Noise is conditioned RMS before conservative post-response ADC quantization.'
  pNearContact : object (value not decoded)
  pNoSprings : object (value not decoded)
  pRecommended : object (value not decoded)
undefined symbols (not defined in the file): DiscIntNeverNeededParam
(part 1 of 3)
settings Model: Creator=tommie  LastModifiedBy=tommie
settings DebuggingCC: AlgebraicLoopMsg=error

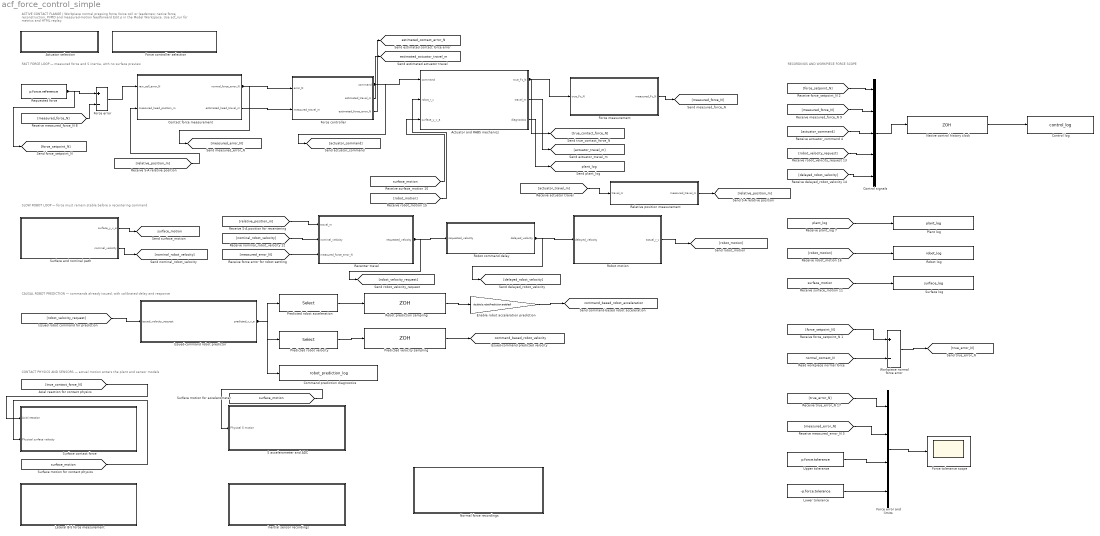
== system acf_force_control_simple ==
  note: ACTIVE CONTACT FLANGE | Workpiece normal pressing force
      | Voice coil or leadscrew; native force reconstruction, PI/PID and measured-motion feedforward
      | Edit p in the Model Workspace. Use acf_run for metrics and HTML replay.
  note: FAST FORCE LOOP — measured force and S inertia, with no surface preview
  note: SLOW ROBOT LOOP — force must remain stable before a recentering command
  note: CAUSAL ROBOT PREDICTION — commands already issued, with calibrated delay and response
  note: CONTACT PHYSICS AND SENSORS — actual motion enters the plant and sensor models
  note: RECORDINGS AND WORKPIECE FORCE SCOPE
  Actuator and RABS mechanics : Subsystem
  Actuator selection : Subsystem  mask(Active contact flange actuator selection){ActuatorChoice=Voice coil}
      mask prompts: ActuatorChoice "Actuator"
      mask help: Choose the motor before running. Mechanical, surface and sensor settings are preserved. Force-controller gains, command units and initial holding current are recalculated for the selected drive.
      mask TypeOptions ActuatorChoice: Leadscrew | Voice coil | Ideal position (reference)
      mask Callback ActuatorChoice: acf_select_actuator(bdroot(gcb),get_param(gcb,'ActuatorChoice'));
      mask Display: disp(sprintf('Actuator selection\n%s',get_param(gcb,'ActuatorChoice')));
  Command prediction diagnostics : ToWorkspace  VariableName=robot_prediction_log  SaveFormat=Timeseries  SampleTime=p.sim.step
  Contact force measurement : Subsystem
  Control log : ToWorkspace  VariableName=control_log  SaveFormat=Timeseries  SampleTime=p.sim.step
  Control signals : Mux  Inputs=5
  Enable robot acceleration prediction : Gain  Gain=double(p.robotPrediction.enabled)
  Force controller : Subsystem  Variant=on  VariantControlMode=label  LabelModeActiveChoice=Coil PI and PID
  Force controller selection : Subsystem  mask{ControllerChoice=Feedforward PI}
      mask prompts: ControllerChoice "Normal force controller"
      mask help: Choose Feedforward PI for the tested controller, or compare PI/PID using the same reconstructed workpiece normal force. Gains live in p.inertial for the coil and p.screw for the leadscrew.
      mask TypeOptions ControllerChoice: Feedforward PI | PI | PID
      mask Callback ControllerChoice: acf_select_controller(bdroot);
      mask Display: disp(sprintf('Normal force control\n%s',get_param(gcb,'ControllerChoice')));
  Force error : Sum  Inputs=+-
  Force error and limits : Mux
  Force measurement : Subsystem
  Force tolerance scope : Scope
  Inertial sensor recordings : Subsystem
  Issued-command robot predictor : Subsystem
  Lateral B-S force measurement : Subsystem
  Lower tolerance : Constant  Value=-p.force.tolerance
  Native control history clock : ZeroOrderHold  SampleTime=p.sim.step
  Normal force recordings : Subsystem
  Plant log : ToWorkspace  VariableName=plant_log  SaveFormat=Timeseries  SampleTime=p.sim.step
  Predicted robot acceleration : Selector  InputPortWidth=3  IndexOptions=Index vector (dialog)  Indices=3  OutputSizes=1
  Predicted robot velocity : Selector  InputPortWidth=3  IndexOptions=Index vector (dialog)  Indices=2  OutputSizes=1
  Predicted velocity sampling : ZeroOrderHold  SampleTime=p.force.sampleTime
  Recenter travel : Subsystem
  Relative position measurement : Subsystem
  Requested force : Constant  Value=p.force.reference
  Robot command delay : Subsystem
  Robot log : ToWorkspace  VariableName=robot_log  SaveFormat=Timeseries  SampleTime=p.sim.step
  Robot motion : Subsystem
  Robot prediction sampling : ZeroOrderHold  SampleTime=p.force.sampleTime
  S accelerometer and ADC : Subsystem
  Surface and nominal path : Subsystem
  Surface contact force : Subsystem
  Surface log : ToWorkspace  VariableName=surface_log  SaveFormat=Timeseries  SampleTime=p.sim.step
  Upper tolerance : Constant  Value=p.force.tolerance
  Workpiece normal force error : Sum  Inputs=+-
  tag scope: command_based_robot_acceleration=global, command_based_robot_velocity=global, estimated_actuator_travel_m=global, estimated_contact_error_N=global, plant_log=global, surface_motion=global
  wires:
  [robot_motion] -> Actuator and RABS mechanics/2(robot_r_v)
  [surface_motion] -> Actuator and RABS mechanics/3(surface_y_v_a)
  [force_setpoint_N] -> Control signals/1
  [measured_force_N] -> Control signals/2
  [actuator_command] -> Control signals/3
  [robot_velocity_request] -> Control signals/4
  [delayed_robot_velocity] -> Control signals/5
  Requested force/1 -> Force error/1, [force_setpoint_N]
  [measured_force_N] -> Force error/2
  [true_error_N] -> Force error and limits/1
  [measured_error_N] -> Force error and limits/2
  Upper tolerance/1 -> Force error and limits/3
  Lower tolerance/1 -> Force error and limits/4
  Actuator and RABS mechanics/1(true_Fc_N) -> [true_contact_force_N], Force measurement/1(true_Fc_N)
  Force error and limits/1 -> Force tolerance scope/1
  [plant_log] -> Plant log/1
  [relative_position_m] -> Recenter travel/1(travel_m)
  [nominal_robot_velocity] -> Recenter travel/2(nominal_velocity)
  Recenter travel/1(requested_velocity) -> [robot_velocity_request], Robot command delay/1(requested_velocity)
  [robot_motion] -> Robot log/1
  Actuator and RABS mechanics/2(travel_m) -> [actuator_travel_m]
  Surface and nominal path/2(nominal_velocity) -> [nominal_robot_velocity]
  Actuator and RABS mechanics/3(diagnostics) -> [plant_log]
  Robot motion/1(actual_r_v) -> [robot_motion]
  Surface and nominal path/1(surface_y_v_a) -> [surface_motion]
  Workpiece normal force error/1 -> [true_error_N]
  [surface_motion] -> Surface log/1
  [force_setpoint_N] -> Workpiece normal force error/1
  [normal_contact_N] -> Workpiece normal force error/2
  Force controller/1(command) -> Actuator and RABS mechanics/1(command), [actuator_command]
  [measured_error_N] -> Recenter travel/3(measured_force_error_N)
  Force controller/2(estimated_travel_m) -> [estimated_actuator_travel_m]
  Force controller/3(estimated_force_error_N) -> [estimated_contact_error_N]
  [robot_velocity_request] -> Issued-command robot predictor/1(issued_velocity_request)
  Issued-command robot predictor/1(predicted_r_v_a) -> Command prediction diagnostics/1, Predicted robot velocity/1, Predicted robot acceleration/1
  Predicted robot acceleration/1 -> Robot prediction sampling/1
  Robot prediction sampling/1 -> Enable robot acceleration prediction/1
  Enable robot acceleration prediction/1 -> [command_based_robot_acceleration]
  Predicted robot velocity/1 -> Predicted velocity sampling/1
  Predicted velocity sampling/1 -> [command_based_robot_velocity]
  Force measurement/1(measured_Fc_N) -> [measured_force_N]
  [actuator_travel_m] -> Relative position measurement/1(travel_m)
  Relative position measurement/1(measured_travel_m) -> [relative_position_m]
  Force error/1 -> Contact force measurement/1(raw_cell_error_N)
  [relative_position_m] -> Contact force measurement/2(measured_head_position_m)
  Contact force measurement/1(normal_force_error_N) -> Force controller/1(error_N), [measured_error_N]
  Contact force measurement/2(estimated_head_travel_m) -> Force controller/2(measured_travel_m)
  Robot command delay/1(delayed_velocity) -> Robot motion/1(delayed_velocity), [delayed_robot_velocity]
  Control signals/1 -> Native control history clock/1
  Native control history clock/1 -> Control log/1
  [true_contact_force_N] -> Surface contact force/1(Axial reaction)
  [surface_motion] -> Surface contact force/2(Physical surface velocity)
  [surface_motion] -> S accelerometer and ADC/1(Physical S motion)

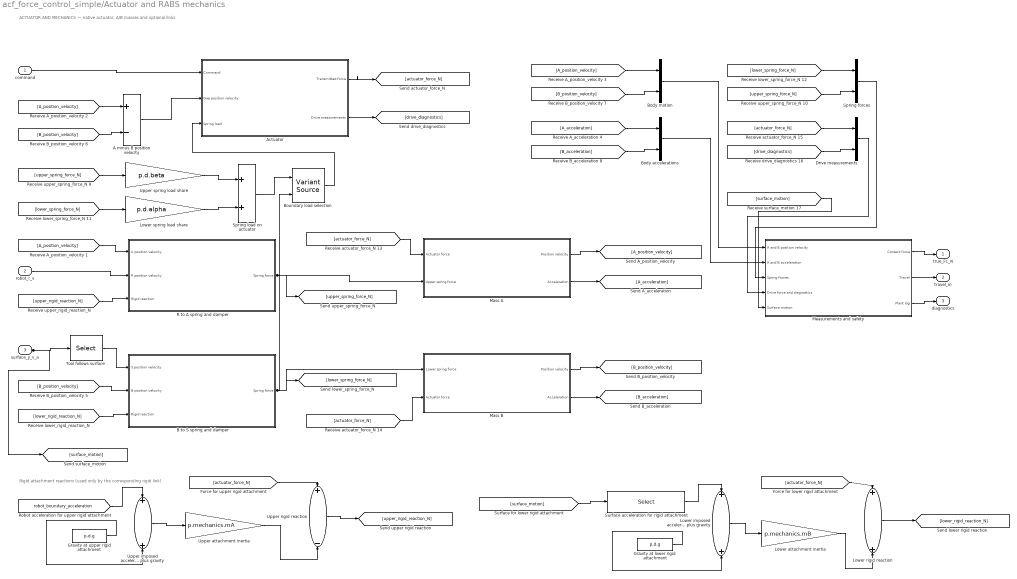
== system acf_force_control_simple/Actuator and RABS mechanics ==
  note: ACTUATOR AND MECHANICS — native actuator, A/B masses and optional links
  note: Rigid attachment reactions (used only by the corresponding rigid link)
  command : Inport
  robot_r_v : Inport  Port=2
  surface_y_v_a : Inport  Port=3
  A minus B position velocity : Sum  Inputs=+-
  Actuator : Subsystem  Variant=on  VariantControlMode=label  LabelModeActiveChoice=Voice coil  PropagateVariantConditions=on
  B to S spring and damper : Subsystem
  Body accelerations : Mux  Inputs=2
  Body motion : Mux  Inputs=2
  Boundary load selection : VariantSource  VariantControlMode=label  LabelModeActiveChoice=Compliant A  VariantControls={Compliant A, Rigid A}
  Drive measurements : Mux  Inputs=2
  Gravity at lower rigid attachment : Constant  Value=p.d.g
  Gravity at upper rigid attachment : Constant  Value=p.d.g
  Lower attachment inertia : Gain  Gain=p.mechanics.mB
  Lower imposed acceleration plus gravity : Sum
  Lower rigid reaction : Sum
  Lower spring load share : Gain  Gain=p.d.alpha
  Mass A : Subsystem
  Mass B : Subsystem
  Measurements and safety : Subsystem
  R to A spring and damper : Subsystem
  Spring forces : Mux  Inputs=2
  Spring load on actuator : Sum
  Surface acceleration for rigid attachment : Selector  InputPortWidth=3  IndexOptions=Index vector (dialog)  Indices=3  OutputSizes=1
  Tool follows surface : Selector  InputPortWidth=3  IndexOptions=Index vector (dialog)  Indices=[1 2]  OutputSizes=1
  Upper attachment inertia : Gain  Gain=p.mechanics.mA
  Upper imposed acceleration plus gravity : Sum
  Upper rigid reaction : Sum  Inputs=+-
  Upper spring load share : Gain  Gain=p.d.beta
  true_Fc_N : Outport
  travel_m : Outport  Port=2
  diagnostics : Outport  Port=3
  wires:
  Mass B/2(Acceleration) -> [B_acceleration]
  Mass B/1(Position velocity) -> [B_position_velocity]
  command/1 -> Actuator/1(Command)
  Upper rigid reaction/1 -> [upper_rigid_reaction_N]
  Actuator/2(Drive measurements) -> [drive_diagnostics]
  B to S spring and damper/1(Spring force) -> Boundary load selection/2, [lower_spring_force_N], Mass B/1(Lower spring force)
  [A_position_velocity] -> A minus B position velocity/1
  Mass A/1(Position velocity) -> [A_position_velocity]
  Measurements and safety/3(Plant log) -> diagnostics/1
  Lower imposed acceleration plus gravity/1 -> Lower attachment inertia/1
  Measurements and safety/2(Travel) -> travel_m/1
  [B_position_velocity] -> B to S spring and damper/2(B position velocity)
  Tool follows surface/1 -> B to S spring and damper/1(S position velocity)
  [A_acceleration] -> Body accelerations/1
  Mass A/2(Acceleration) -> [A_acceleration]
  [A_position_velocity] -> R to A spring and damper/1(A position velocity)
  [A_position_velocity] -> Body motion/1
  [lower_spring_force_N] -> Spring forces/1
  [actuator_force_N] -> Drive measurements/1
  Actuator/1(Transmitted force) -> [actuator_force_N]
  Body motion/1 -> Measurements and safety/1(A and B position velocity)
  Lower attachment inertia/1 -> Lower rigid reaction/2
  [actuator_force_N] -> Upper rigid reaction/1
  [B_position_velocity] -> Body motion/2
  robot_r_v/1 -> R to A spring and damper/2(R position velocity)
  [upper_spring_force_N] -> Spring forces/2
  [surface_motion] -> Surface acceleration for rigid attachment/1
  [B_position_velocity] -> A minus B position velocity/2
  surface_y_v_a/1 -> Tool follows surface/1, [surface_motion]
  A minus B position velocity/1 -> Actuator/2(Gap position velocity)
  [actuator_force_N] -> Lower rigid reaction/1
  Surface acceleration for rigid attachment/1 -> Lower imposed acceleration plus gravity/1
  Upper imposed acceleration plus gravity/1 -> Upper attachment inertia/1
  [actuator_force_N] -> Mass B/2(Actuator force)
  Spring load on actuator/1 -> Boundary load selection/1
  Upper attachment inertia/1 -> Upper rigid reaction/2
  [B_acceleration] -> Body accelerations/2
  Gravity at lower rigid attachment/1 -> Lower imposed acceleration plus gravity/2
  Lower spring load share/1 -> Spring load on actuator/2
  [lower_rigid_reaction_N] -> B to S spring and damper/3(Rigid reaction)
  [upper_rigid_reaction_N] -> R to A spring and damper/3(Rigid reaction)
  Gravity at upper rigid attachment/1 -> Upper imposed acceleration plus gravity/2
  [lower_spring_force_N] -> Lower spring load share/1
  Boundary load selection/1 -> Actuator/3(Spring load)
  Measurements and safety/1(Contact force) -> true_Fc_N/1
  [drive_diagnostics] -> Drive measurements/2
  Body accelerations/1 -> Measurements and safety/2(A and B acceleration)
  Lower rigid reaction/1 -> [lower_rigid_reaction_N]
  Drive measurements/1 -> Measurements and safety/4(Drive force and diagnostics)
  [surface_motion] -> Measurements and safety/5(Surface motion)
  [upper_spring_force_N] -> Upper spring load share/1
  [actuator_force_N] -> Mass A/1(Actuator force)
  Spring forces/1 -> Measurements and safety/3(Spring forces)
  R to A spring and damper/1(Spring force) -> [upper_spring_force_N], Mass A/2(Upper spring force)
  [robot_boundary_acceleration] -> Upper imposed acceleration plus gravity/1
  Upper spring load share/1 -> Spring load on actuator/1

== system acf_force_control_simple/Actuator selection ==

== system acf_force_control_simple/Contact force measurement ==
  raw_cell_error_N : Inport
  measured_head_position_m : Inport  Port=2
  Contact force reconstruction : Subsystem
  Head motion estimator : Subsystem
  Normal force error sign : Gain  Gain=-1
  Normal force projection : Subsystem
  normal_force_error_N : Outport
  estimated_head_travel_m : Outport  Port=2
  tag scope: inertial_axial_reference_deviation_N=global, inertial_head_gap_velocity=global
  wires:
  Normal force error sign/1 -> normal_force_error_N/1
  Normal force projection/2(axial_reference_deviation_N) -> [inertial_axial_reference_deviation_N]
  Normal force projection/1(normal_force_deviation_N) -> Normal force error sign/1
  Contact force reconstruction/1(axial_contact_N) -> Normal force projection/1(Compensated axial force)
  Head motion estimator/2(estimated_head_travel_m) -> estimated_head_travel_m/1
  Head motion estimator/1(head_gap_velocity_m_s) -> [inertial_head_gap_velocity], Normal force projection/3(Head gap velocity)
  raw_cell_error_N/1 -> Contact force reconstruction/1(raw_cell_error_N)
  Contact force reconstruction/2(lateral_contact_N) -> Normal force projection/2(Compensated lateral force)
  measured_head_position_m/1 -> Head motion estimator/1(measured_head_position_m)

== system acf_force_control_simple/Force controller ==
  error_N : Inport
  measured_travel_m : Inport  Port=2
  Coil PI and PID : Subsystem  VariantControl=Coil PI and PID
  Drive PI and PID : Subsystem  VariantControl=Drive PI and PID
  Screw normal PI and PID : Subsystem  VariantControl=Screw normal PI and PID
  command : Outport
  estimated_travel_m : Outport  Port=2
  estimated_force_error_N : Outport  Port=3

== system acf_force_control_simple/Force controller selection ==

== system acf_force_control_simple/Force measurement ==
  note: PHYSICAL SENSOR AND KNOWN-WEIGHT TARE
      | Cell between B and S: raw cell = Fc - mS*(gravity + tool acceleration).
      | Tare removes mS*gravity; motion inertia remains in the sampled force reading.
      | The physical acceleration above models the load cell. The controller never receives it.
      | Set distalMass_kg = 0 only for the near-contact reference.
  note: Compensated force channel
      | Sampling + filter + bias + noise + delay
      | Numerical step p.sim.step; sampling periods are independent.
  true_Fc_N : Inport
  Axial gravity : Constant  Value=p.d.g
  Conditioned force with tare residual : Sum
  Engineered common AA and EMA : DiscreteTransferFcn  Numerator=p.d.acquisition.responses.force.numerator  Denominator=p.d.acquisition.responses.force.denominator  InitialStates=(p.force.reference)*p.d.acquisition.responses.force.steadyStatePerUnitInput  SampleTime=p.sensor.sampleTime
  Fresh 10 kHz force frame : ZeroOrderHold  SampleTime=p.force.sampleTime
  Known downstream tool mass : Gain  Gain=p.sensor.distalMass_kg
  Known weight tare : Constant  Value=p.sensor.distalMass_kg*p.d.g
  Physical B-S load cell : Sum  Inputs=+-
  Physical tool acceleration : Selector  InputPortWidth=3  IndexOptions=Index vector (dialog)  Indices=3  OutputSizes=1
  Raw noisy force sample : Sum
  Raw output-noise normalization : Gain  Gain=p.d.acquisition.noiseInputScale
  Sensor bias : Constant  Value=p.sensor.bias
  Sensor noise RMS : Gain  Gain=p.sensor.noiseRms
  Sensor sample delay : Delay  DelayLength=p.d.sensorDelaySamples  InitialCondition=p.force.reference+p.sensor.bias  SampleTime=p.sensor.sampleTime
  Sensor sampling : ZeroOrderHold  SampleTime=p.sensor.sampleTime
  Tared cell force : Sum
  Tool specific acceleration : Sum
  Uniform sensor noise : UniformRandomNumber  Minimum=-sqrt(3)  Maximum=sqrt(3)  Seed=p.sensor.seed  SampleTime=p.sensor.sampleTime
  measured_Fc_N : Outport
  wires:
  Sensor bias/1 -> Conditioned force with tare residual/2
  Engineered common AA and EMA/1 -> Conditioned force with tare residual/1
  Raw output-noise normalization/1 -> Raw noisy force sample/2
  Sensor sampling/1 -> Raw noisy force sample/1
  [surface_motion] -> Physical tool acceleration/1
  true_Fc_N/1 -> Physical B-S load cell/1
  Sensor sample delay/1 -> Fresh 10 kHz force frame/1
  Known weight tare/1 -> Tared cell force/2
  Raw noisy force sample/1 -> Engineered common AA and EMA/1
  [downstream_force_N] -> Physical B-S load cell/2
  Tared cell force/1 -> Sensor sampling/1
  Fresh 10 kHz force frame/1 -> measured_Fc_N/1
  Sensor noise RMS/1 -> Raw output-noise normalization/1
  Physical tool acceleration/1 -> Tool specific acceleration/1
  Axial gravity/1 -> Tool specific acceleration/2
  Physical B-S load cell/1 -> Tared cell force/1
  Uniform sensor noise/1 -> Sensor noise RMS/1
  Tool specific acceleration/1 -> Known downstream tool mass/1
  Conditioned force with tare residual/1 -> Sensor sample delay/1
  Known downstream tool mass/1 -> [downstream_force_N]

== system acf_force_control_simple/Inertial sensor recordings ==
  Acceleration and reconstructed force : Mux  Inputs=6
  Acceleration validation log : ToWorkspace  VariableName=accelerometer_log  SaveFormat=Timeseries  SampleTime=p.sim.step
  Head motion recording clock : ZeroOrderHold  SampleTime=p.sim.step
  Motion observer validation log : ToWorkspace  VariableName=inertial_motion_log  SaveFormat=Timeseries  SampleTime=p.sim.step
  Record every physical step {1..6} (6 alike) : ZeroOrderHold  SampleTime=p.sim.step
  wires:
  Acceleration and reconstructed force/1 -> Acceleration validation log/1
  Head motion recording clock/1 -> Motion observer validation log/1
  [measured_S_acceleration_z] -> Record every physical step 1/1
  [measured_S_acceleration_x] -> Record every physical step 2/1
  [inertial_lateral_contact_N] -> Record every physical step 6/1
  Record every physical step 1/1 -> Acceleration and reconstructed force/1
  [physical_S_acceleration_z] -> Record every physical step 3/1
  Record every physical step 5/1 -> Acceleration and reconstructed force/5
  [physical_S_acceleration_x] -> Record every physical step 4/1
  Record every physical step 6/1 -> Acceleration and reconstructed force/6
  [inertial_axial_contact_N] -> Record every physical step 5/1
  [inertial_head_motion_states] -> Head motion recording clock/1
  Record every physical step 4/1 -> Acceleration and reconstructed force/4
  Record every physical step 3/1 -> Acceleration and reconstructed force/3
  Record every physical step 2/1 -> Acceleration and reconstructed force/2

== system acf_force_control_simple/Issued-command robot predictor ==
  issued_velocity_request : Inport
  Expected acceleration limit : Saturate  UpperLimit=p.robotPrediction.maxAcceleration  LowerLimit=-p.robotPrediction.maxAcceleration
  Expected command delay : Delay  DelayLength=p.robotPrediction.delaySamples  InitialCondition=p.robot.nominalVelocity*double(~p.robotPrediction.boundedNominalPath)  SampleTime=p.robot.sampleTime
  Expected speed limit : Saturate  UpperLimit=p.robotPrediction.maxSpeed  LowerLimit=-p.robotPrediction.maxSpeed
  Expected velocity response : Gain  Gain=1/p.robotPrediction.responseTime
  Predicted position velocity acceleration : Mux  Inputs=3
  Predicted relative position : Integrator
  Predicted velocity : Integrator
  Predicted velocity error : Sum  Inputs=+-
  predicted_r_v_a : Outport
  wires:
  Predicted position velocity acceleration/1 -> predicted_r_v_a/1
  Predicted relative position/1 -> Predicted position velocity acceleration/1
  Predicted velocity/1 -> [prediction_internal_velocity], Predicted relative position/1, Predicted position velocity acceleration/2
  Expected acceleration limit/1 -> Predicted velocity/1, Predicted position velocity acceleration/3
  Expected velocity response/1 -> Expected acceleration limit/1
  Predicted velocity error/1 -> Expected velocity response/1
  Expected speed limit/1 -> Predicted velocity error/1
  Expected command delay/1 -> Expected speed limit/1
  [prediction_internal_velocity] -> Predicted velocity error/2
  issued_velocity_request/1 -> Expected command delay/1

== system acf_force_control_simple/Lateral B-S force measurement ==
  Conditioned force with tare residual : Sum
  Engineered common AA and EMA : DiscreteTransferFcn  Numerator=p.d.acquisition.responses.lateral.numerator  Denominator=p.d.acquisition.responses.lateral.denominator  InitialStates=(-p.force.reference*p.contact.mu)*p.d.acquisition.responses.lateral.steadyStatePerUnitInput  SampleTime=p.sensor.sampleTime
  Filtered derivative memory : Gain  Gain=exp(-p.sensor.sampleTime/p.contact.lateralDerivativeFilterTime_s)
  Filtered derivative new sample : Gain  Gain=(1-exp(-p.sensor.sampleTime/p.contact.lateralDerivativeFilterTime_s))/p.sensor.sampleTime
  Filtered lateral force derivative : Sum
  Fresh 10 kHz force frame : ZeroOrderHold  SampleTime=p.force.sampleTime
  Identified lateral latency : Gain  Gain=p.contact.lateralPredictionTime_s
  Independent lateral noise : UniformRandomNumber  Minimum=-sqrt(3)  Maximum=sqrt(3)  Seed=p.sensor.seed+197  SampleTime=p.sensor.sampleTime
  Known tare residual bias : Constant  Value=p.contact.lateralBias_N
  Measured lateral force increment : Sum  Inputs=+-
  Noise RMS : Gain  Gain=p.contact.lateralNoiseRms_N
  Present lateral force estimate : Sum
  Previous lateral derivative : UnitDelay  SampleTime=p.sensor.sampleTime
  Previous measured lateral force : UnitDelay  InitialCondition=-p.force.reference*p.contact.mu  SampleTime=p.sensor.sampleTime
  Raw noisy force sample : Sum
  Raw output-noise normalization : Gain  Gain=p.d.acquisition.noiseInputScale
  Sensor sample delay : Delay  DelayLength=p.contact.lateralDelaySamples  InitialCondition=-p.force.reference*p.contact.mu  SampleTime=p.sensor.sampleTime
  Sensor sampling : ZeroOrderHold  SampleTime=p.sensor.sampleTime
  tag scope: measured_lateral_contact_N=global, predicted_lateral_contact_N=global
  wires:
  Identified lateral latency/1 -> Present lateral force estimate/2
  Present lateral force estimate/1 -> [predicted_lateral_contact_N]
  Filtered lateral force derivative/1 -> Identified lateral latency/1, Previous lateral derivative/1
  Filtered derivative new sample/1 -> Filtered lateral force derivative/1
  Previous lateral derivative/1 -> Filtered derivative memory/1
  Previous measured lateral force/1 -> Measured lateral force increment/2
  Independent lateral noise/1 -> Noise RMS/1
  Sensor sampling/1 -> Raw noisy force sample/1
  [lateral_contact_N] -> Sensor sampling/1
  Engineered common AA and EMA/1 -> Conditioned force with tare residual/1
  Measured lateral force increment/1 -> Filtered derivative new sample/1
  Conditioned force with tare residual/1 -> Sensor sample delay/1
  Sensor sample delay/1 -> Fresh 10 kHz force frame/1
  Raw output-noise normalization/1 -> Raw noisy force sample/2
  Fresh 10 kHz force frame/1 -> [measured_lateral_contact_N], Measured lateral force increment/1, Previous measured lateral force/1, Present lateral force estimate/1
  Raw noisy force sample/1 -> Engineered common AA and EMA/1
  Filtered derivative memory/1 -> Filtered lateral force derivative/2
  Noise RMS/1 -> Raw output-noise normalization/1
  Known tare residual bias/1 -> Conditioned force with tare residual/2

== system acf_force_control_simple/Normal force recordings ==
  Normal logging sample {1..8} (8 alike) : ZeroOrderHold  SampleTime=p.sim.step
  Surface normal diagnostics : Mux  Inputs=8
  Surface normal log : ToWorkspace  VariableName=normal_contact_log  SaveFormat=Timeseries  SampleTime=p.sim.step
  wires:
  Surface normal diagnostics/1 -> Surface normal log/1
  Normal logging sample 8/1 -> Surface normal diagnostics/8
  Normal logging sample 6/1 -> Surface normal diagnostics/6
  [normal_contact_N] -> Normal logging sample 1/1
  [measured_lateral_contact_N] -> Normal logging sample 7/1
  [command_based_robot_velocity] -> Normal logging sample 8/1
  Normal logging sample 2/1 -> Surface normal diagnostics/2
  [estimated_contact_slope] -> Normal logging sample 5/1
  [estimated_normal_contact_N] -> Normal logging sample 4/1
  Normal logging sample 1/1 -> Surface normal diagnostics/1
  [actual_contact_slope] -> Normal logging sample 3/1
  [requested_axial_contact_N] -> Normal logging sample 6/1
  Normal logging sample 3/1 -> Surface normal diagnostics/3
  Normal logging sample 4/1 -> Surface normal diagnostics/4
  Normal logging sample 7/1 -> Surface normal diagnostics/7
  [lateral_contact_N] -> Normal logging sample 2/1
  Normal logging sample 5/1 -> Surface normal diagnostics/5

== system acf_force_control_simple/Recenter travel ==
  note: Mid-stroke - actual travel
      | Deadband + slow gain + nominal robot path
      | Numerical step p.sim.step; sampling periods are independent.
  travel_m : Inport
  nominal_velocity : Inport  Port=2
  measured_force_error_N : Inport  Port=3
  Distance from mid stroke : Sum  Inputs=+-
  Force settling gate : Subsystem
  Gate contact or cell error : Switch  Criteria=u2 ~= 0  SaturateOnIntegerOverflow=off  InputSameDT=off
  Hold recentering : Constant  Value=0
  Measured or estimated travel : Switch  Criteria=u2 ~= 0  SaturateOnIntegerOverflow=off  InputSameDT=off
  Mid stroke : Constant  Value=p.mechanics.midTravel
  Nominal path sampling : ZeroOrderHold  SampleTime=p.robot.sampleTime
  Recenter deadband : DeadZone  LowerValue=-p.robot.deadband  UpperValue=p.robot.deadband
  Recenter gain : Gain  Gain=p.d.recenterGain
  Robot feedback sampling : ZeroOrderHold  SampleTime=p.robot.sampleTime
  Robot speed limits : Saturate  UpperLimit=p.robot.maxSpeed  LowerLimit=-p.robot.maxSpeed
  Robot velocity request : Sum
  Send correction only when settled : Switch  Threshold=.5  SaturateOnIntegerOverflow=off  InputSameDT=off
  Tool sensor needs gap estimate : Constant  Value=p.sensor.positionModel
  Use reconstructed contact error : Constant  Value=double(p.sensor.distalMass_kg>0 && strcmp(p.actuator.kind,'voice_coil') && strcmp(p.coil.strategy,'observer'))
  requested_velocity : Outport
  wires:
  Send correction only when settled/1 -> Robot velocity request/2
  Hold recentering/1 -> Send correction only when settled/3
  Robot velocity request/1 -> Robot speed limits/1
  Force settling gate/1(ready) -> Send correction only when settled/2
  Recenter gain/1 -> Send correction only when settled/1
  Gate contact or cell error/1 -> Force settling gate/1(force_error_N)
  nominal_velocity/1 -> Nominal path sampling/1
  Tool sensor needs gap estimate/1 -> Measured or estimated travel/2
  travel_m/1 -> Measured or estimated travel/3
  [estimated_actuator_travel_m] -> Measured or estimated travel/1
  Nominal path sampling/1 -> [nominal_velocity]
  measured_force_error_N/1 -> Gate contact or cell error/3
  Measured or estimated travel/1 -> Robot feedback sampling/1
  Mid stroke/1 -> Distance from mid stroke/1
  Use reconstructed contact error/1 -> Gate contact or cell error/2
  Robot feedback sampling/1 -> Distance from mid stroke/2
  Distance from mid stroke/1 -> Recenter deadband/1
  [nominal_velocity] -> Robot velocity request/1
  [estimated_contact_error_N] -> Gate contact or cell error/1
  Robot speed limits/1 -> requested_velocity/1
  Recenter deadband/1 -> Recenter gain/1

== system acf_force_control_simple/Relative position measurement ==
  travel_m : Inport
  Coordinate reference : Constant  Value=p.mechanics.midTravel
  Measurement delay : Delay  DelayLength=p.d.strokeDelaySamples  InitialCondition=p.d.positionMeasurementInitial  SampleTime=p.d.positionSampleTime
  Position noise : UniformRandomNumber  Minimum=-sqrt(3)  Maximum=sqrt(3)  Seed=p.sensor.seed+1  SampleTime=p.d.positionSampleTime
  Position noise RMS : Gain  Gain=p.sensor.strokeNoiseRms*p.d.acquisition.positionNoiseInputScale
  Position sampling : ZeroOrderHold  SampleTime=p.d.positionSampleTime
  Select A and S : Selector  InputPortWidth=25  IndexOptions=Index vector (dialog)  Indices=[5 7]  OutputSizes=1
  Select position instrument : Switch  Criteria=u2 ~= 0  SaturateOnIntegerOverflow=off  InputSameDT=off
  Sensed position : Sum
  Tool S relative to A : Gain  Gain=[-1 1]  Multiplication=Matrix(K*u)
  Tool measurement coordinate : Sum
  Use toolhead position : Constant  Value=p.sensor.positionModel
  measured_travel_m : Outport
  wires:
  Measurement delay/1 -> measured_travel_m/1
  Position noise RMS/1 -> Sensed position/2
  Position sampling/1 -> Sensed position/1
  Position noise/1 -> Position noise RMS/1
  Select position instrument/1 -> Position sampling/1
  Sensed position/1 -> Measurement delay/1
  travel_m/1 -> Select position instrument/3
  Use toolhead position/1 -> Select position instrument/2
  Tool S relative to A/1 -> Tool measurement coordinate/1
  Coordinate reference/1 -> Tool measurement coordinate/2
  Select A and S/1 -> Tool S relative to A/1
  Tool measurement coordinate/1 -> Select position instrument/1
  [plant_log] -> Select A and S/1

== system acf_force_control_simple/Robot command delay ==
  note: Delay measured in robot command samples
      | Numerical step p.sim.step; sampling periods are independent.
  requested_velocity : Inport
  Held issued command at transport clock : ZeroOrderHold  SampleTime=p.d.actualRobotTransportSampleTime_s
  Robot command samples : Delay  DelayLength=p.d.robotDelaySamples  InitialCondition=p.robot.nominalVelocity*double(~p.robotPrediction.boundedNominalPath)  SampleTime=p.d.actualRobotTransportSampleTime_s
  delayed_velocity : Outport
  wires:
  Held issued command at transport clock/1 -> Robot command samples/1
  Robot command samples/1 -> delayed_velocity/1
  requested_velocity/1 -> Held issued command at transport clock/1

== system acf_force_control_simple/Robot motion ==
  note: Velocity response + speed/acceleration limits
      | Prescribed robot boundary, no robot force input
      | Numerical step p.sim.step; sampling periods are independent.
  delayed_velocity : Inport
  Requested robot speed : Saturate  UpperLimit=p.robot.maxSpeed  LowerLimit=-p.robot.maxSpeed
  Robot acceleration limits : Saturate  UpperLimit=p.robot.maxAcceleration  LowerLimit=-p.robot.maxAcceleration
  Robot position : Integrator  InitialCondition=p.d.r0
  Robot position and velocity : Mux  Inputs=2
  Robot speed error : Sum  Inputs=+-
  Robot velocity : Integrator
  Velocity response : Gain  Gain=1/p.robot.responseTime
  actual_r_v : Outport
  tag scope: robot_boundary_acceleration=global
  wires:
  Robot velocity/1 -> [robot_velocity_m_s], Robot position/1
  Robot acceleration limits/1 -> [robot_boundary_acceleration], Robot velocity/1
  Velocity response/1 -> Robot acceleration limits/1
  Robot position/1 -> [robot_position_m]
  Robot speed error/1 -> Velocity response/1
  [robot_velocity_m_s] -> Robot speed error/2
  Robot position and velocity/1 -> actual_r_v/1
  Requested robot speed/1 -> Robot speed error/1
  [robot_velocity_m_s] -> Robot position and velocity/2
  delayed_velocity/1 -> Requested robot speed/1
  [robot_position_m] -> Robot position and velocity/1

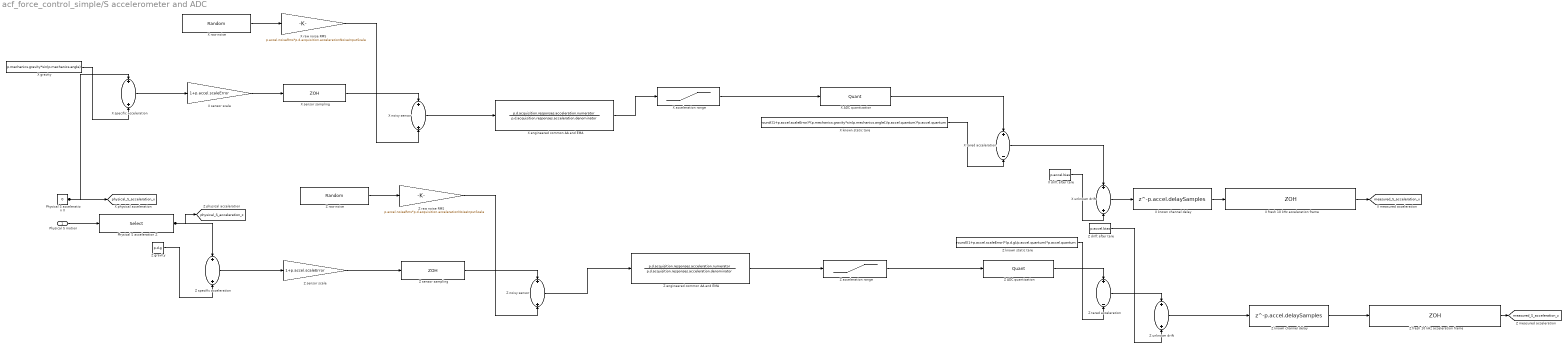
== system acf_force_control_simple/S accelerometer and ADC ==
  Physical S motion : Inport
  Physical S acceleration X : Constant  Value=0
  Physical S acceleration Z : Selector  InputPortWidth=3  IndexOptions=Index vector (dialog)  Indices=3  OutputSizes=1
  X ADC quantization : Quantizer  QuantizationInterval=p.accel.quantum
  X acceleration range : Saturate  UpperLimit=p.accel.range_g*p.mechanics.gravity  LowerLimit=-p.accel.range_g*p.mechanics.gravity
  X drift after tare : Constant  Value=p.accel.bias
  X engineered common AA and EMA : DiscreteTransferFcn  Numerator=p.d.acquisition.responses.acceleration.numerator  Denominator=p.d.acquisition.responses.acceleration.denominator  InitialStates=((1+p.accel.scaleError)*(p.mechanics.gravity*sin(p.mechanics.angle)))*p.d.acquisition.responses.acceleration.steadyStatePerUnitInput  SampleTime=p.sensor.sampleTime
  X fresh 10 kHz acceleration frame : ZeroOrderHold  SampleTime=p.force.sampleTime
  X gravity : Constant  Value=p.mechanics.gravity*sin(p.mechanics.angle)
  X known channel delay : Delay  DelayLength=p.accel.delaySamples  InitialCondition=p.accel.bias  SampleTime=p.sensor.sampleTime
  X known static tare : Constant  Value=round((1+p.accel.scaleError)*(p.mechanics.gravity*sin(p.mechanics.angle))/p.accel.quantum)*p.accel.quantum
  X noisy sensor : Sum
  X raw noise : RandomNumber  Seed=p.sensor.seed+336  SampleTime=p.sensor.sampleTime
  X raw noise RMS : Gain  Gain=p.accel.noiseRms*p.d.acquisition.accelerationNoiseInputScale
  X sensor sampling : ZeroOrderHold  SampleTime=p.sensor.sampleTime
  X sensor scale : Gain  Gain=1+p.accel.scaleError
  X specific acceleration : Sum
  X tared acceleration : Sum  Inputs=+-
  X unknown drift : Sum
  Z ADC quantization : Quantizer  QuantizationInterval=p.accel.quantum
  Z acceleration range : Saturate  UpperLimit=p.accel.range_g*p.mechanics.gravity  LowerLimit=-p.accel.range_g*p.mechanics.gravity
  Z drift after tare : Constant  Value=p.accel.bias
  Z engineered common AA and EMA : DiscreteTransferFcn  Numerator=p.d.acquisition.responses.acceleration.numerator  Denominator=p.d.acquisition.responses.acceleration.denominator  InitialStates=((1+p.accel.scaleError)*(p.d.g))*p.d.acquisition.responses.acceleration.steadyStatePerUnitInput  SampleTime=p.sensor.sampleTime
  Z fresh 10 kHz acceleration frame : ZeroOrderHold  SampleTime=p.force.sampleTime
  Z gravity : Constant  Value=p.d.g
  Z known channel delay : Delay  DelayLength=p.accel.delaySamples  InitialCondition=p.accel.bias  SampleTime=p.sensor.sampleTime
  Z known static tare : Constant  Value=round((1+p.accel.scaleError)*(p.d.g)/p.accel.quantum)*p.accel.quantum
  Z noisy sensor : Sum
  Z raw noise : RandomNumber  Seed=p.sensor.seed+239  SampleTime=p.sensor.sampleTime
  Z raw noise RMS : Gain  Gain=p.accel.noiseRms*p.d.acquisition.accelerationNoiseInputScale
  Z sensor sampling : ZeroOrderHold  SampleTime=p.sensor.sampleTime
  Z sensor scale : Gain  Gain=1+p.accel.scaleError
  Z specific acceleration : Sum
  Z tared acceleration : Sum  Inputs=+-
  Z unknown drift : Sum
  tag scope: measured_S_acceleration_x=global, measured_S_acceleration_z=global, physical_S_acceleration_x=global, physical_S_acceleration_z=global
  wires:
  X fresh 10 kHz acceleration frame/1 -> [measured_S_acceleration_x]
  X known channel delay/1 -> X fresh 10 kHz acceleration frame/1
  Z tared acceleration/1 -> Z unknown drift/1
  Z drift after tare/1 -> Z unknown drift/2
  Z unknown drift/1 -> Z known channel delay/1
  X unknown drift/1 -> X known channel delay/1
  Z fresh 10 kHz acceleration frame/1 -> [measured_S_acceleration_z]
  X drift after tare/1 -> X unknown drift/2
  X tared acceleration/1 -> X unknown drift/1
  X sensor scale/1 -> X sensor sampling/1
  Z specific acceleration/1 -> Z sensor scale/1
  X specific acceleration/1 -> X sensor scale/1
  Physical S acceleration Z/1 -> [physical_S_acceleration_z], Z specific acceleration/1
  X acceleration range/1 -> X ADC quantization/1
  Physical S motion/1 -> Physical S acceleration Z/1
  X gravity/1 -> X specific acceleration/2
  X raw noise/1 -> X raw noise RMS/1
  Z acceleration range/1 -> Z ADC quantization/1
  Z raw noise/1 -> Z raw noise RMS/1
  X sensor sampling/1 -> X noisy sensor/1
  Z sensor scale/1 -> Z sensor sampling/1
  X engineered common AA and EMA/1 -> X acceleration range/1
  X noisy sensor/1 -> X engineered common AA and EMA/1
  Z gravity/1 -> Z specific acceleration/2
  Z known static tare/1 -> Z tared acceleration/2
  Z raw noise RMS/1 -> Z noisy sensor/2
  X ADC quantization/1 -> X tared acceleration/1
  Z sensor sampling/1 -> Z noisy sensor/1
  Physical S acceleration X/1 -> [physical_S_acceleration_x], X specific acceleration/1
  Z noisy sensor/1 -> Z engineered common AA and EMA/1
  Z known channel delay/1 -> Z fresh 10 kHz acceleration frame/1
  Z engineered common AA and EMA/1 -> Z acceleration range/1
  X known static tare/1 -> X tared acceleration/2
  X raw noise RMS/1 -> X noisy sensor/2
  Z ADC quantization/1 -> Z tared acceleration/1

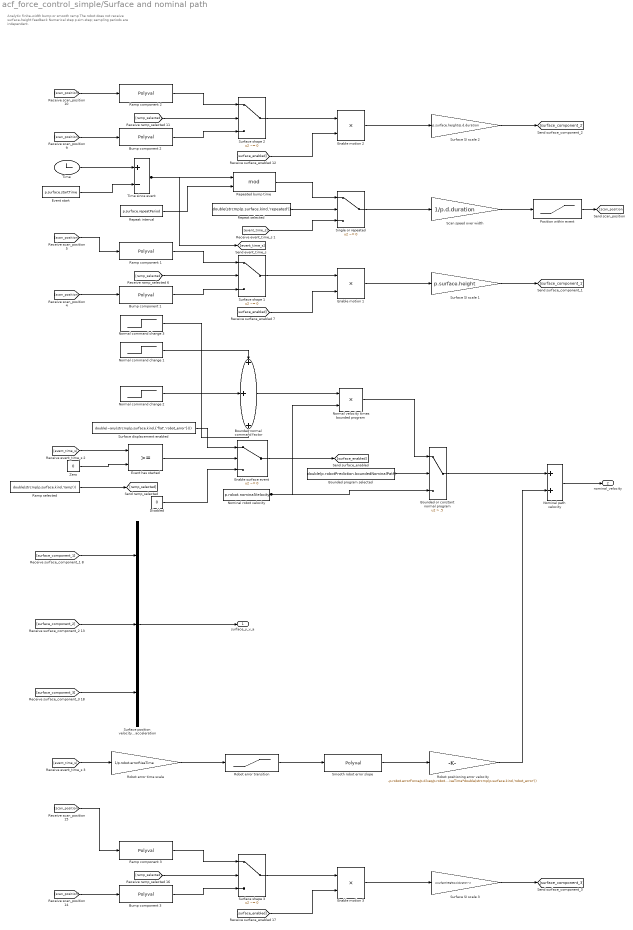
== system acf_force_control_simple/Surface and nominal path ==
  note: Analytic finite-width bump or smooth ramp
      | The robot does not receive surface-height feedback
      | Numerical step p.sim.step; sampling periods are independent.
  Bounded normal command factor : Sum  Inputs=+++
  Bounded or constant normal program : Switch  Criteria=u2 > Threshold  Threshold=.5  SaturateOnIntegerOverflow=off  InputSameDT=off
  Bounded program selected : Constant  Value=double(p.robotPrediction.boundedNominalPath)
  Bump component 1 : Polyval  Coefs=[-64 192 -192 64 0 0 0]
  Bump component 2 : Polyval  Coefs=[-384 960 -768 192 0 0]
  Bump component 3 : Polyval  Coefs=[-1920 3840 -2304 384 0]
  Disabled : Constant  Value=0
  Enable motion 1 : Product
  Enable motion 2 : Product
  Enable motion 3 : Product
  Enable surface event : Switch  Criteria=u2 ~= 0  SaturateOnIntegerOverflow=off  InputSameDT=off
  Event has started : RelationalOperator  OutDataTypeStr=boolean  RndMeth=Simplest  InputSameDT=off
  Event start : Constant  Value=p.surface.startTime
  Nominal path velocity : Sum
  Nominal robot velocity : Constant  Value=p.robot.nominalVelocity
  Normal command change 1 : Step  SampleTime=p.robot.sampleTime
  Normal command change 2 : Step  Time=2  FinalValue=-2  SampleTime=p.robot.sampleTime
  Normal command change 3 : Step  Time=3  SampleTime=p.robot.sampleTime
  Normal velocity times bounded program : Product
  Position within event : Saturate  UpperLimit=1  LowerLimit=0
  Ramp component 1 : Polyval  Coefs=[6 -15 10 0 0 0]
  Ramp component 2 : Polyval  Coefs=[30 -60 30 0 0]
  Ramp component 3 : Polyval  Coefs=[120 -180 60 0]
  Ramp selected : Constant  Value=double(strcmp(p.surface.kind,'ramp'))
  Repeat interval : Constant  Value=p.surface.repeatPeriod
  Repeat selected : Constant  Value=double(strcmp(p.surface.kind,'repeated'))
  Repeated bump time : Math  Operator=mod
  Robot error time scale : Gain  Gain=1/p.robot.errorRiseTime
  Robot error transition : Saturate  UpperLimit=1  LowerLimit=0
  Robot positioning error velocity : Gain  Gain=-p.robot.errorForce/p.d.keq/p.robot.errorRiseTime*double(strcmp(p.surface.kind,'robot_error'))
  Scan speed over width : Gain  Gain=1/p.d.duration
  Single or repeated : Switch  Criteria=u2 ~= 0  SaturateOnIntegerOverflow=off  InputSameDT=off
  Smooth robot error slope : Polyval  Coefs=[30 -60 30 0 0]
  Surface SI scale 1 : Gain  Gain=p.surface.height
  Surface SI scale 2 : Gain  Gain=p.surface.height/p.d.duration
  Surface SI scale 3 : Gain  Gain=p.surface.height/p.d.duration^2
  Surface displacement enabled : Constant  Value=double(~any(strcmp(p.surface.kind,{'flat','robot_error'})))
  Surface position velocity acceleration : Mux  Inputs=3
  Surface shape 1 : Switch  Criteria=u2 ~= 0  SaturateOnIntegerOverflow=off  InputSameDT=off
  Surface shape 2 : Switch  Criteria=u2 ~= 0  SaturateOnIntegerOverflow=off  InputSameDT=off
  Surface shape 3 : Switch  Criteria=u2 ~= 0  SaturateOnIntegerOverflow=off  InputSameDT=off
  Time : Clock
  Time since event : Sum  Inputs=+-
  Zero : Constant  Value=0
  surface_y_v_a : Outport
  nominal_velocity : Outport  Port=2
  wires:
  Nominal path velocity/1 -> nominal_velocity/1
  Surface SI scale 3/1 -> [surface_component_3]
  Normal command change 1/1 -> Bounded normal command factor/1
  Repeat interval/1 -> Repeated bump time/2
  Normal command change 2/1 -> Bounded normal command factor/2
  [surface_component_2] -> Surface position velocity acceleration/2
  Repeat selected/1 -> Single or repeated/2
  Time since event/1 -> [event_time_s], Repeated bump time/1
  Bump component 2/1 -> Surface shape 2/3
  [ramp_selected] -> Surface shape 1/2
  Robot error transition/1 -> Smooth robot error slope/1
  [scan_position] -> Bump component 3/1
  Event has started/1 -> Enable surface event/2
  Surface shape 1/1 -> Enable motion 1/1
  Enable motion 1/1 -> Surface SI scale 1/1
  Event start/1 -> Time since event/2
  Normal velocity times bounded program/1 -> Bounded or constant normal program/1
  [scan_position] -> Ramp component 3/1
  [scan_position] -> Ramp component 2/1
  Normal command change 3/1 -> Bounded normal command factor/3
  Position within event/1 -> [scan_position]
  [ramp_selected] -> Surface shape 3/2
  Time/1 -> Time since event/1
  [event_time_s] -> Event has started/1
  Zero/1 -> Event has started/2
  Repeated bump time/1 -> Single or repeated/1
  Bump component 1/1 -> Surface shape 1/3
  [scan_position] -> Bump component 2/1
  Disabled/1 -> Enable surface event/3
  Bounded normal command factor/1 -> Normal velocity times bounded program/1
  [ramp_selected] -> Surface shape 2/2
  Robot positioning error velocity/1 -> Nominal path velocity/2
  Ramp component 1/1 -> Surface shape 1/1
  [surface_enabled] -> Enable motion 3/2
  Ramp selected/1 -> [ramp_selected]
  [surface_component_1] -> Surface position velocity acceleration/1
  [surface_component_3] -> Surface position velocity acceleration/3
  [scan_position] -> Ramp component 1/1
  [event_time_s] -> Robot error time scale/1
  Robot error time scale/1 -> Robot error transition/1
  [surface_enabled] -> Enable motion 1/2
  Ramp component 3/1 -> Surface shape 3/1
  Surface position velocity acceleration/1 -> surface_y_v_a/1
  Surface SI scale 2/1 -> [surface_component_2]
  Bump component 3/1 -> Surface shape 3/3
  Surface shape 2/1 -> Enable motion 2/1
  Surface SI scale 1/1 -> [surface_component_1]
  [surface_enabled] -> Enable motion 2/2
  [event_time_s] -> Single or repeated/3
  Enable surface event/1 -> [surface_enabled]
  Surface shape 3/1 -> Enable motion 3/1
  Enable motion 2/1 -> Surface SI scale 2/1
  Single or repeated/1 -> Scan speed over width/1
  Surface displacement enabled/1 -> Enable surface event/1
  Nominal robot velocity/1 -> Normal velocity times bounded program/2, Bounded or constant normal program/3
  Bounded program selected/1 -> Bounded or constant normal program/2
  Smooth robot error slope/1 -> Robot positioning error velocity/1
  Enable motion 3/1 -> Surface SI scale 3/1
  Ramp component 2/1 -> Surface shape 2/1
  Scan speed over width/1 -> Position within event/1
  [scan_position] -> Bump component 1/1
  Bounded or constant normal program/1 -> Nominal path velocity/1

== system acf_force_control_simple/Surface contact force ==
  Axial reaction : Inport
  Physical surface velocity : Inport  Port=2
  Axial reaction factor : Sum  Inputs=+-
  Friction times slope : Gain  Gain=p.contact.mu
  Lateral reaction : Product  Inputs=**/
  Lateral sign : Gain  Gain=-1
  Normal reaction : Product  Inputs=**/
  Normalizer : Math  Operator=sqrt
  Slope plus friction : Bias  Bias=p.contact.mu  SaturateOnIntegerOverflow=off
  Squared slope : Math  Operator=square
  Squared slope plus one : Bias  Bias=1  SaturateOnIntegerOverflow=off
  Surface slope : Gain  Gain=1/p.surface.scanSpeed
  Unity : Constant
  Velocity component : Selector  InputPortWidth=3  IndexOptions=Index vector (dialog)  Indices=2  OutputSizes=1
  tag scope: actual_contact_slope=global, lateral_contact_N=global, normal_contact_N=global
  wires:
  Lateral sign/1 -> [lateral_contact_N]
  Velocity component/1 -> Surface slope/1
  Physical surface velocity/1 -> Velocity component/1
  Surface slope/1 -> [actual_contact_slope], Squared slope/1, Friction times slope/1, Slope plus friction/1
  Lateral reaction/1 -> Lateral sign/1
  Unity/1 -> Axial reaction factor/1
  Friction times slope/1 -> Axial reaction factor/2
  Squared slope/1 -> Squared slope plus one/1
  Axial reaction factor/1 -> Normal reaction/3
  Axial reaction/1 -> Normal reaction/1
  Squared slope plus one/1 -> Normalizer/1
  Normalizer/1 -> Normal reaction/2, Lateral reaction/3
  Normal reaction/1 -> [normal_contact_N], Lateral reaction/1
  Slope plus friction/1 -> Lateral reaction/2

== system acf_force_control_simple/Actuator and RABS mechanics/Actuator ==
  Command : Inport
  Gap position velocity : Inport  Port=2
  Spring load : Inport  Port=3
  Ideal position : Subsystem  VariantControl=Ideal position
  Leadscrew : Subsystem  VariantControl=Leadscrew
  Voice coil : Subsystem  VariantControl=Voice coil
  Transmitted force : Outport
  Drive measurements : Outport  Port=2

== system acf_force_control_simple/Actuator and RABS mechanics/B to S spring and damper ==
  S position velocity : Inport
  B position velocity : Inport  Port=2
  Rigid reaction : Inport  Port=3
  Compliant or rigid link : VariantSource  VariantControlMode=label  LabelModeActiveChoice=Compliant  VariantControls={Compliant, Rigid}
  Damping : Gain  Gain=p.mechanics.c1
  Endpoint difference : Sum  Inputs=+-
  Preload : Constant  Value=p.d.q10
  Spring and damper force : Sum  Inputs=+++
  Spring displacement and relative velocity : Demux  Outputs=2
  Stiffness : Gain  Gain=p.mechanics.k1
  Spring force : Outport
  wires:
  Compliant or rigid link/1 -> Spring force/1
  Rigid reaction/1 -> Compliant or rigid link/2
  Spring and damper force/1 -> Compliant or rigid link/1
  Damping/1 -> Spring and damper force/3
  Stiffness/1 -> Spring and damper force/2
  Spring displacement and relative velocity/2 -> Damping/1
  Preload/1 -> Spring and damper force/1
  Spring displacement and relative velocity/1 -> Stiffness/1
  Endpoint difference/1 -> Spring displacement and relative velocity/1
  B position velocity/1 -> Endpoint difference/2
  S position velocity/1 -> Endpoint difference/1

== system acf_force_control_simple/Actuator and RABS mechanics/Mass A ==
  Actuator force : Inport
  Upper spring force : Inport  Port=2
  Gravity : Constant  Value=p.d.g
  Inverse mass : Gain  Gain=1/p.mechanics.mA
  Net applied force : Sum  Inputs=+-
  Newton acceleration : Sum  Inputs=+-
  Position : Integrator  InitialCondition=p.d.u0
  Position and velocity : Mux  Inputs=2
  Velocity : Integrator
  Position velocity : Outport
  Acceleration : Outport  Port=2
  wires:
  [velocity_m_s] -> Position and velocity/2
  Velocity/1 -> [velocity_m_s], Position/1
  Newton acceleration/1 -> Acceleration/1, Velocity/1
  Gravity/1 -> Newton acceleration/2
  Position and velocity/1 -> Position velocity/1
  Position/1 -> Position and velocity/1
  Inverse mass/1 -> Newton acceleration/1
  Net applied force/1 -> Inverse mass/1
  Upper spring force/1 -> Net applied force/2
  Actuator force/1 -> Net applied force/1

== system acf_force_control_simple/Actuator and RABS mechanics/Mass B ==
  Lower spring force : Inport
  Actuator force : Inport  Port=2
  Gravity : Constant  Value=p.d.g
  Inverse mass : Gain  Gain=1/p.mechanics.mB
  Net applied force : Sum  Inputs=+-
  Newton acceleration : Sum  Inputs=+-
  Position : Integrator
  Position and velocity : Mux  Inputs=2
  Velocity : Integrator
  Position velocity : Outport
  Acceleration : Outport  Port=2
  wires:
  Position and velocity/1 -> Position velocity/1
  [velocity_m_s] -> Position and velocity/2
  Position/1 -> Position and velocity/1
  Velocity/1 -> [velocity_m_s], Position/1
  Newton acceleration/1 -> Acceleration/1, Velocity/1
  Inverse mass/1 -> Newton acceleration/1
  Net applied force/1 -> Inverse mass/1
  Actuator force/1 -> Net applied force/2
  Gravity/1 -> Newton acceleration/2
  Lower spring force/1 -> Net applied force/1
